simulink model "rfdc"  (R2019a)
settings: Solver=VariableStepAuto  StartTime=0.0  StopTime=10.0  RelTol=1e-3
libraries: xbsIndex_r4 x6
(part 1 of 2)
settings Model: Creator=mcb  LastModifiedBy=bjacobm

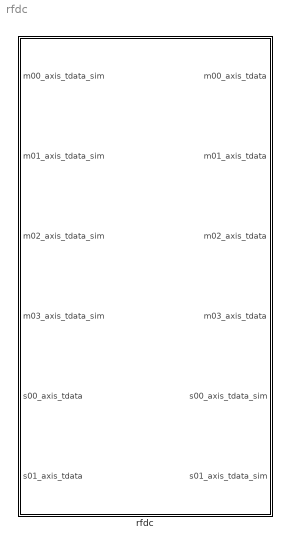
== system rfdc ==
  rfdc : Subsystem  Tag=xps:rfdc  mask(Xilinx RF Data Converter){forceredraw=0, maskopening=1, runinit=1, Tile224_enable=on, t224_enable_mts=off, t224_sample_rate=2000, t224_clk_out=125, t224_enable_pll=on, t224_ref_clk=250, t224_axi_stream_clk=[], t224_QT_adc0_enable=on, t224_QT_adc0_digital_output=I/Q, t224_QT_adc0_dec_mode=4x, t224_QT_adc0_sample_per_cycle=4, t224_QT_adc0_req_axis_clk=250, t224_QT_adc0_mixer_type=Fine, t224_QT_adc0_mixer_mode=Real -> I/Q, t224_QT_adc0_nco_freq=0, t224_QT_adc0_nco_phase=0, t224_QT_adc0_coarse_freq=0, t224_QT_adc0_nyquist_zone=Zone 1, t224_QT_adc0_cal_mode=Mode 2, t224_QT_adc1_enable=on, t224_QT_adc1_digital_output=I/Q, t224_QT_adc1_dec_mode=4x, t224_QT_adc1_sample_per_cycle=4, t224_QT_adc1_req_axis_clk=250, t224_QT_adc1_mixer_type=Fine, t224_QT_adc1_mixer_mode=Real -> I/Q, t224_QT_adc1_nco_freq=0, t224_QT_adc1_nco_phase=0, t224_QT_adc1_coarse_freq=0, t224_QT_adc1_nyquist_zone=Zone 1, t224_QT_adc1_cal_mode=Mode 2, t224_QT_adc2_enable=on, t224_QT_adc2_digital_output=I/Q, t224_QT_adc2_dec_mode=4x, t224_QT_adc2_sample_per_cycle=4, t224_QT_adc2_req_axis_clk=250, t224_QT_adc2_mixer_type=Fine, t224_QT_adc2_mixer_mode=Real -> I/Q, t224_QT_adc2_nco_freq=0, t224_QT_adc2_nco_phase=0, t224_QT_adc2_coarse_freq=0, t224_QT_adc2_nyquist_zone=Zone 1, t224_QT_adc2_cal_mode=Mode 2, t224_QT_adc3_enable=on, t224_QT_adc3_digital_output=I/Q, t224_QT_adc3_dec_mode=4x, t224_QT_adc3_sample_per_cycle=4, t224_QT_adc3_req_axis_clk=250, t224_QT_adc3_mixer_type=Fine, t224_QT_adc3_mixer_mode=Real -> I/Q, t224_QT_adc3_nco_freq=0, t224_QT_adc3_nco_phase=0, t224_QT_adc3_coarse_freq=0, t224_QT_adc3_nyquist_zone=Zone 1, t224_QT_adc3_cal_mode=Mode 2, t224_DT_adc0_enable=on, t224_DT_adc0_digital_output=Real, t224_DT_adc0_dec_mode=2x, t224_DT_adc0_sample_per_cycle=8, t224_DT_adc0_req_axis_clk=125, t224_DT_adc0_mixer_type=Bypassed, t224_DT_adc0_mixer_mode=Real -> Real, t224_DT_adc0_nco_freq=0, t224_DT_adc0_nco_phase=0, t224_DT_adc0_coarse_freq=0, t224_DT_adc0_nyquist_zone=Zone 1, t224_DT_adc0_cal_mode=Mode 2, t224_DT_adc1_enable=on, t224_DT_adc1_digital_output=Real, t224_DT_adc1_dec_mode=2x, t224_DT_adc1_sample_per_cycle=8, t224_DT_adc1_req_axis_clk=125, t224_DT_adc1_mixer_type=Bypassed, t224_DT_adc1_mixer_mode=Real -> Real, t224_DT_adc1_nco_freq=0, t224_DT_adc1_nco_phase=0, t224_DT_adc1_coarse_freq=0, t224_DT_adc1_nyquist_zone=Zone 1, t224_DT_adc1_cal_mode=Mode 2, Tile225_enable=off, t225_enable_mts=off, t225_sample_rate=2000, t225_clk_out=125, t225_enable_pll=on, t225_ref_clk=250, t225_axi_stream_clk=[], t225_QT_adc0_enable=on, t225_QT_adc0_digital_output=Real, t225_QT_adc0_dec_mode=4x, t225_QT_adc0_sample_per_cycle=2, t225_QT_adc0_req_axis_clk=250, t225_QT_adc0_mixer_type=Bypassed, t225_QT_adc0_mixer_mode=Real -> Real, t225_QT_adc0_nco_freq=0, t225_QT_adc0_nco_phase=0, t225_QT_adc0_coarse_freq=0, t225_QT_adc0_nyquist_zone=Zone 1, t225_QT_adc0_cal_mode=Mode 2, t225_QT_adc1_enable=off, t225_QT_adc1_digital_output=Real, t225_QT_adc1_dec_mode=4x, t225_QT_adc1_sample_per_cycle=2, t225_QT_adc1_req_axis_clk=250, t225_QT_adc1_mixer_type=Bypassed, t225_QT_adc1_mixer_mode=Real -> Real, t225_QT_adc1_nco_freq=0, t225_QT_adc1_nco_phase=0, t225_QT_adc1_coarse_freq=0, t225_QT_adc1_nyquist_zone=Zone 1, t225_QT_adc1_cal_mode=Mode 2, t225_QT_adc2_enable=off, t225_QT_adc2_digital_output=Real, t225_QT_adc2_dec_mode=4x, t225_QT_adc2_sample_per_cycle=2, t225_QT_adc2_req_axis_clk=250, t225_QT_adc2_mixer_type=Bypassed, t225_QT_adc2_mixer_mode=Real -> Real, t225_QT_adc2_nco_freq=0, t225_QT_adc2_nco_phase=0, t225_QT_adc2_coarse_freq=0, t225_QT_adc2_nyquist_zone=Zone 1, t225_QT_adc2_cal_mode=Mode 2, t225_QT_adc3_enable=off, t225_QT_adc3_digital_output=Real, t225_QT_adc3_dec_mode=4x, t225_QT_adc3_sample_per_cycle=2, t225_QT_adc3_req_axis_clk=250, t225_QT_adc3_mixer_type=Bypassed, t225_QT_adc3_mixer_mode=Real -> Real, t225_QT_adc3_nco_freq=0, t225_QT_adc3_nco_phase=0, t225_QT_adc3_coarse_freq=0, t225_QT_adc3_nyquist_zone=Zone 1, t225_QT_adc3_cal_mode=Mode 2, t225_DT_adc0_enable=on, t225_DT_adc0_digital_output=Real, t225_DT_adc0_dec_mode=2x, t225_DT_adc0_sample_per_cycle=8, t225_DT_adc0_req_axis_clk=125, t225_DT_adc0_mixer_type=Bypassed, t225_DT_adc0_mixer_mode=Real -> Real, t225_DT_adc0_nco_freq=0, t225_DT_adc0_nco_phase=0, t225_DT_adc0_coarse_freq=0, t225_DT_adc0_nyquist_zone=Zone 1, t225_DT_adc0_cal_mode=Mode 2, t225_DT_adc1_enable=on, t225_DT_adc1_digital_output=Real, t225_DT_adc1_dec_mode=2x, t225_DT_adc1_sample_per_cycle=8, t225_DT_adc1_req_axis_clk=125, t225_DT_adc1_mixer_type=Bypassed, t225_DT_adc1_mixer_mode=Real -> Real, t225_DT_adc1_nco_freq=0, t225_DT_adc1_nco_phase=0, t225_DT_adc1_coarse_freq=0, t225_DT_adc1_nyquist_zone=Zone 1, t225_DT_adc1_cal_mode=Mode 2, Tile226_enable=off, t226_enable_mts=off, t226_sample_rate=2000, t226_clk_out=125, t226_enable_pll=on, t226_ref_clk=250, t226_axi_stream_clk=[], t226_QT_adc0_enable=on, t226_QT_adc0_digital_output=Real, t226_QT_adc0_dec_mode=4x, t226_QT_adc0_sample_per_cycle=2, t226_QT_adc0_req_axis_clk=250, t226_QT_adc0_mixer_type=Bypassed, t226_QT_adc0_mixer_mode=Real -> Real, t226_QT_adc0_nco_freq=0, t226_QT_adc0_nco_phase=0, t226_QT_adc0_coarse_freq=0, t226_QT_adc0_nyquist_zone=Zone 1, t226_QT_adc0_cal_mode=Mode 2, t226_QT_adc1_enable=off, t226_QT_adc1_digital_output=Real, t226_QT_adc1_dec_mode=4x, t226_QT_adc1_sample_per_cycle=2, t226_QT_adc1_req_axis_clk=250, t226_QT_adc1_mixer_type=Bypassed, t226_QT_adc1_mixer_mode=Real -> Real, t226_QT_adc1_nco_freq=0, t226_QT_adc1_nco_phase=0, t226_QT_adc1_coarse_freq=0, t226_QT_adc1_nyquist_zone=Zone 1, t226_QT_adc1_cal_mode=Mode 2, t226_QT_adc2_enable=off, t226_QT_adc2_digital_output=Real, t226_QT_adc2_dec_mode=4x, t226_QT_adc2_sample_per_cycle=2, t226_QT_adc2_req_axis_clk=250, t226_QT_adc2_mixer_type=Bypassed, t226_QT_adc2_mixer_mode=Real -> Real, t226_QT_adc2_nco_freq=0, t226_QT_adc2_nco_phase=0, t226_QT_adc2_coarse_freq=0, t226_QT_adc2_nyquist_zone=Zone 1, t226_QT_adc2_cal_mode=Mode 2, t226_QT_adc3_enable=off, t226_QT_adc3_digital_output=Real, t226_QT_adc3_dec_mode=4x, t226_QT_adc3_sample_per_cycle=2, t226_QT_adc3_req_axis_clk=250, t226_QT_adc3_mixer_type=Bypassed, t226_QT_adc3_mixer_mode=Real -> Real, t226_QT_adc3_nco_freq=0, t226_QT_adc3_nco_phase=0, t226_QT_adc3_coarse_freq=0, t226_QT_adc3_nyquist_zone=Zone 1, t226_QT_adc3_cal_mode=Mode 2, t226_DT_adc0_enable=on, t226_DT_adc0_digital_output=Real, t226_DT_adc0_dec_mode=2x, t226_DT_adc0_sample_per_cycle=8, t226_DT_adc0_req_axis_clk=125, t226_DT_adc0_mixer_type=Bypassed, t226_DT_adc0_mixer_mode=Real -> Real, t226_DT_adc0_nco_freq=0, t226_DT_adc0_nco_phase=0, t226_DT_adc0_coarse_freq=0, t226_DT_adc0_nyquist_zone=Zone 1, t226_DT_adc0_cal_mode=Mode 2, t226_DT_adc1_enable=on, t226_DT_adc1_digital_output=Real, t226_DT_adc1_dec_mode=2x, t226_DT_adc1_sample_per_cycle=8, t226_DT_adc1_req_axis_clk=125, t226_DT_adc1_mixer_type=Bypassed, t226_DT_adc1_mixer_mode=Real -> Real, t226_DT_adc1_nco_freq=0, t226_DT_adc1_nco_phase=0, t226_DT_adc1_coarse_freq=0, t226_DT_adc1_nyquist_zone=Zone 1, t226_DT_adc1_cal_mode=Mode 2, Tile227_enable=off, t227_enable_mts=off, t227_sample_rate=2000, t227_clk_out=125, t227_enable_pll=on, t227_ref_clk=250, t227_axi_stream_clk=[], t227_QT_adc0_enable=on, t227_QT_adc0_digital_output=Real, t227_QT_adc0_dec_mode=4x, t227_QT_adc0_sample_per_cycle=2, t227_QT_adc0_req_axis_clk=250, t227_QT_adc0_mixer_type=Bypassed, t227_QT_adc0_mixer_mode=Real -> Real, t227_QT_adc0_nco_freq=0, t227_QT_adc0_nco_phase=0, t227_QT_adc0_coarse_freq=0, t227_QT_adc0_nyquist_zone=Zone 1, t227_QT_adc0_cal_mode=Mode 2, t227_QT_adc1_enable=off, t227_QT_adc1_digital_output=Real, t227_QT_adc1_dec_mode=4x, t227_QT_adc1_sample_per_cycle=2, t227_QT_adc1_req_axis_clk=250, t227_QT_adc1_mixer_type=Bypassed, t227_QT_adc1_mixer_mode=Real -> Real, t227_QT_adc1_nco_freq=0, t227_QT_adc1_nco_phase=0, t227_QT_adc1_coarse_freq=0, t227_QT_adc1_nyquist_zone=Zone 1, t227_QT_adc1_cal_mode=Mode 2, t227_QT_adc2_enable=off, t227_QT_adc2_digital_output=Real, t227_QT_adc2_dec_mode=4x, t227_QT_adc2_sample_per_cycle=2, t227_QT_adc2_req_axis_clk=250, t227_QT_adc2_mixer_type=Bypassed, t227_QT_adc2_mixer_mode=Real -> Real, t227_QT_adc2_nco_freq=0, t227_QT_adc2_nco_phase=0, t227_QT_adc2_coarse_freq=0, t227_QT_adc2_nyquist_zone=Zone 1, t227_QT_adc2_cal_mode=Mode 2, t227_QT_adc3_enable=off, t227_QT_adc3_digital_output=Real, t227_QT_adc3_dec_mode=4x, t227_QT_adc3_sample_per_cycle=2, t227_QT_adc3_req_axis_clk=250, t227_QT_adc3_mixer_type=Bypassed, t227_QT_adc3_mixer_mode=Real -> Real, t227_QT_adc3_nco_freq=0, t227_QT_adc3_nco_phase=0, t227_QT_adc3_coarse_freq=0, t227_QT_adc3_nyquist_zone=Zone 1, t227_QT_adc3_cal_mode=Mode 2, t227_DT_adc0_enable=on, t227_DT_adc0_digital_output=Real, t227_DT_adc0_dec_mode=2x, t227_DT_adc0_sample_per_cycle=8, t227_DT_adc0_req_axis_clk=125, t227_DT_adc0_mixer_type=Bypassed, t227_DT_adc0_mixer_mode=Real -> Real, t227_DT_adc0_nco_freq=0, t227_DT_adc0_nco_phase=0, t227_DT_adc0_coarse_freq=0, t227_DT_adc0_nyquist_zone=Zone 1, t227_DT_adc0_cal_mode=Mode 2, t227_DT_adc1_enable=on, t227_DT_adc1_digital_output=Real, t227_DT_adc1_dec_mode=2x, t227_DT_adc1_sample_per_cycle=8, t227_DT_adc1_req_axis_clk=125, t227_DT_adc1_mixer_type=Bypassed, t227_DT_adc1_mixer_mode=Real -> Real, t227_DT_adc1_nco_freq=0, t227_DT_adc1_nco_phase=0, t227_DT_adc1_coarse_freq=0, t227_DT_adc1_nyquist_zone=Zone 1, t227_DT_adc1_cal_mode=Mode 2, Tile228_enable=on, t228_enable_mts=off, t228_sample_rate=2000, t228_clk_out=125, t228_enable_pll=on, t228_ref_clk=250, t228_axi_stream_clk=[], t228_output_power=20, t228_QT_dac0_enable=on, t228_QT_dac0_analog_output=Real, t228_QT_dac0_inter_mode=4x, t228_QT_dac0_sample_per_cycle=2, t228_QT_dac0_req_axis_clk=250, t228_QT_dac0_datapath_mode=DUC 0 to Fs/2, t228_QT_dac0_mixer_type=Bypassed, t228_QT_dac0_mixer_mode=Real -> Real, t228_QT_dac0_nco_freq=0, t228_QT_dac0_nco_phase=0, t228_QT_dac0_coarse_freq=0, t228_QT_dac0_nyquist_zone=Zone 1, t228_QT_dac0_decode_mode=SNR Optimized, t228_QT_dac1_enable=on, t228_QT_dac1_analog_output=Real, t228_QT_dac1_inter_mode=4x, t228_QT_dac1_sample_per_cycle=2, t228_QT_dac1_req_axis_clk=250, t228_QT_dac1_datapath_mode=DUC 0 to Fs/2, t228_QT_dac1_mixer_type=Bypassed, t228_QT_dac1_mixer_mode=Real -> Real, t228_QT_dac1_nco_freq=0, t228_QT_dac1_nco_phase=0, t228_QT_dac1_coarse_freq=0, t228_QT_dac1_nyquist_zone=Zone 1, t228_QT_dac1_decode_mode=SNR Optimized, t228_QT_dac2_enable=off, t228_QT_dac2_analog_output=Real, t228_QT_dac2_inter_mode=4x, t228_QT_dac2_sample_per_cycle=2, t228_QT_dac2_req_axis_clk=250, t228_QT_dac2_datapath_mode=DUC 0 to Fs/2, t228_QT_dac2_mixer_type=Bypassed, t228_QT_dac2_mixer_mode=Real -> Real, t228_QT_dac2_nco_freq=0, t228_QT_dac2_nco_phase=0, t228_QT_dac2_coarse_freq=0, t228_QT_dac2_nyquist_zone=Zone 1, t228_QT_dac2_decode_mode=SNR Optimized, t228_QT_dac3_enable=off, t228_QT_dac3_analog_output=Real, t228_QT_dac3_inter_mode=4x, t228_QT_dac3_sample_per_cycle=2, t228_QT_dac3_req_axis_clk=250, t228_QT_dac3_datapath_mode=DUC 0 to Fs/2, t228_QT_dac3_mixer_type=Bypassed, t228_QT_dac3_mixer_mode=Real -> Real, t228_QT_dac3_nco_freq=0, t228_QT_dac3_nco_phase=0, t228_QT_dac3_coarse_freq=0, t228_QT_dac3_nyquist_zone=Zone 1, t228_QT_dac3_decode_mode=SNR Optimized, t228_DT_dac0_enable=on, t228_DT_dac0_analog_output=I/Q, t228_DT_dac0_inter_mode=2x, t228_DT_dac0_sample_per_cycle=8, t228_DT_dac0_req_axis_clk=125, t228_DT_dac0_mixer_type=Fine, t228_DT_dac0_mixer_mode=I/Q -> I/Q, t228_DT_dac0_nco_freq=0, t228_DT_dac0_nco_phase=0, t228_DT_dac0_coarse_freq=0, t228_DT_dac0_nyquist_zone=Zone 1, t228_DT_dac0_decode_mode=SNR Optimized, t228_DT_dac1_enable=on, t228_DT_dac1_analog_output=I/Q, t228_DT_dac1_inter_mode=2x, t228_DT_dac1_sample_per_cycle=8, t228_DT_dac1_req_axis_clk=125, t228_DT_dac1_mixer_type=Off, t228_DT_dac1_mixer_mode=Off, t228_DT_dac1_nco_freq=0, t228_DT_dac1_nco_phase=0, t228_DT_dac1_coarse_freq=0, t228_DT_dac1_nyquist_zone=Zone 1, t228_DT_dac1_decode_mode=SNR Optimized, t228_DT_dac2_enable=on, t228_DT_dac2_analog_output=Real, t228_DT_dac2_inter_mode=2x, t228_DT_dac2_sample_per_cycle=8, t228_DT_dac2_req_axis_clk=125, t228_DT_dac2_mixer_type=Bypassed, t228_DT_dac2_mixer_mode=Real -> Real, t228_DT_dac2_nco_freq=0, t228_DT_dac2_nco_phase=0, t228_DT_dac2_coarse_freq=0, t228_DT_dac2_nyquist_zone=Zone 1, t228_DT_dac2_decode_mode=SNR Optimized, t228_DT_dac3_enable=off, t228_DT_dac3_analog_output=Real, t228_DT_dac3_inter_mode=2x, t228_DT_dac3_sample_per_cycle=8, t228_DT_dac3_req_axis_clk=125, t228_DT_dac3_mixer_type=Bypassed, t228_DT_dac3_mixer_mode=Real -> Real, t228_DT_dac3_nco_freq=0, t228_DT_dac3_nco_phase=0, t228_DT_dac3_coarse_freq=0, t228_DT_dac3_nyquist_zone=Zone 1, t228_DT_dac3_decode_mode=SNR Optimized, Tile229_enable=off, t229_enable_mts=off, t229_sample_rate=2000, t229_clk_out=125, t229_enable_pll=on, t229_ref_clk=250, t229_axi_stream_clk=[], t229_output_power=20, t229_QT_dac0_enable=on, t229_QT_dac0_analog_output=Real, t229_QT_dac0_inter_mode=4x, t229_QT_dac0_sample_per_cycle=2, t229_QT_dac0_req_axis_clk=250, t229_QT_dac0_datapath_mode=DUC 0 to Fs/2, t229_QT_dac0_mixer_type=Bypassed, t229_QT_dac0_mixer_mode=Real -> Real, t229_QT_dac0_nco_freq=0, t229_QT_dac0_nco_phase=0, t229_QT_dac0_coarse_freq=0, t229_QT_dac0_nyquist_zone=Zone 1, t229_QT_dac0_decode_mode=SNR Optimized, t229_QT_dac1_enable=off, t229_QT_dac1_analog_output=Real, t229_QT_dac1_inter_mode=4x, t229_QT_dac1_sample_per_cycle=2, t229_QT_dac1_req_axis_clk=250, t229_QT_dac1_datapath_mode=DUC 0 to Fs/2, t229_QT_dac1_mixer_type=Bypassed, t229_QT_dac1_mixer_mode=Real -> Real, t229_QT_dac1_nco_freq=0, t229_QT_dac1_nco_phase=0, t229_QT_dac1_coarse_freq=0, t229_QT_dac1_nyquist_zone=Zone 1, t229_QT_dac1_decode_mode=SNR Optimized, t229_QT_dac2_enable=off, t229_QT_dac2_analog_output=Real, t229_QT_dac2_inter_mode=4x, t229_QT_dac2_sample_per_cycle=2, t229_QT_dac2_req_axis_clk=250, t229_QT_dac2_datapath_mode=DUC 0 to Fs/2, t229_QT_dac2_mixer_type=Bypassed, t229_QT_dac2_mixer_mode=Real -> Real, t229_QT_dac2_nco_freq=0, t229_QT_dac2_nco_phase=0, t229_QT_dac2_coarse_freq=0, t229_QT_dac2_nyquist_zone=Zone 1, t229_QT_dac2_decode_mode=SNR Optimized, t229_QT_dac3_enable=off, t229_QT_dac3_analog_output=Real, t229_QT_dac3_inter_mode=4x, t229_QT_dac3_sample_per_cycle=2, t229_QT_dac3_req_axis_clk=250, t229_QT_dac3_datapath_mode=DUC 0 to Fs/2, t229_QT_dac3_mixer_type=Bypassed, t229_QT_dac3_mixer_mode=Real -> Real, t229_QT_dac3_nco_freq=0, t229_QT_dac3_nco_phase=0, t229_QT_dac3_coarse_freq=0, t229_QT_dac3_nyquist_zone=Zone 1, t229_QT_dac3_decode_mode=SNR Optimized, t229_DT_dac0_enable=off, t229_DT_dac0_analog_output=Real, t229_DT_dac0_inter_mode=2x, t229_DT_dac0_sample_per_cycle=8, t229_DT_dac0_req_axis_clk=125, t229_DT_dac0_mixer_type=Bypassed, t229_DT_dac0_mixer_mode=Real -> Real, t229_DT_dac0_nco_freq=0, t229_DT_dac0_nco_phase=0, t229_DT_dac0_coarse_freq=0, t229_DT_dac0_nyquist_zone=Zone 1, t229_DT_dac0_decode_mode=SNR Optimized, t229_DT_dac1_enable=off, t229_DT_dac1_analog_output=Real, t229_DT_dac1_inter_mode=2x, t229_DT_dac1_sample_per_cycle=8, t229_DT_dac1_req_axis_clk=125, t229_DT_dac1_mixer_type=Bypassed, t229_DT_dac1_mixer_mode=Real -> Real, t229_DT_dac1_nco_freq=0, t229_DT_dac1_nco_phase=0, t229_DT_dac1_coarse_freq=0, t229_DT_dac1_nyquist_zone=Zone 1, t229_DT_dac1_decode_mode=SNR Optimized, t229_DT_dac2_enable=off, t229_DT_dac2_analog_output=Real, t229_DT_dac2_inter_mode=2x, t229_DT_dac2_sample_per_cycle=8, t229_DT_dac2_req_axis_clk=125, t229_DT_dac2_mixer_type=Bypassed, t229_DT_dac2_mixer_mode=Real -> Real, t229_DT_dac2_nco_freq=0, t229_DT_dac2_nco_phase=0, t229_DT_dac2_coarse_freq=0, t229_DT_dac2_nyquist_zone=Zone 1, t229_DT_dac2_decode_mode=SNR Optimized, t229_DT_dac3_enable=off, t229_DT_dac3_analog_output=Real, t229_DT_dac3_inter_mode=2x, t229_DT_dac3_sample_per_cycle=8, t229_DT_dac3_req_axis_clk=125, t229_DT_dac3_mixer_type=Bypassed, t229_DT_dac3_mixer_mode=Real -> Real, t229_DT_dac3_nco_freq=0, t229_DT_dac3_nco_phase=0, t229_DT_dac3_coarse_freq=0, t229_DT_dac3_nyquist_zone=Zone 1, t229_DT_dac3_decode_mode=SNR Optimized, Tile230_enable=off, t230_enable_mts=off, t230_sample_rate=2000, t230_clk_out=125, t230_enable_pll=on, t230_ref_clk=250, t230_axi_stream_clk=[], t230_output_power=20, t230_QT_dac0_enable=on, t230_QT_dac0_analog_output=Real, t230_QT_dac0_inter_mode=4x, t230_QT_dac0_sample_per_cycle=2, t230_QT_dac0_req_axis_clk=250, t230_QT_dac0_datapath_mode=DUC 0 to Fs/2, t230_QT_dac0_mixer_type=Bypassed, t230_QT_dac0_mixer_mode=Real -> Real, t230_QT_dac0_nco_freq=0, t230_QT_dac0_nco_phase=0, t230_QT_dac0_coarse_freq=0, t230_QT_dac0_nyquist_zone=Zone 1, t230_QT_dac0_decode_mode=SNR Optimized, t230_QT_dac1_enable=off, t230_QT_dac1_analog_output=Real, t230_QT_dac1_inter_mode=4x, t230_QT_dac1_sample_per_cycle=2, t230_QT_dac1_req_axis_clk=250, t230_QT_dac1_datapath_mode=DUC 0 to Fs/2, t230_QT_dac1_mixer_type=Bypassed, t230_QT_dac1_mixer_mode=Real -> Real, t230_QT_dac1_nco_freq=0, t230_QT_dac1_nco_phase=0, t230_QT_dac1_coarse_freq=0, t230_QT_dac1_nyquist_zone=Zone 1, t230_QT_dac1_decode_mode=SNR Optimized, t230_QT_dac2_enable=off, t230_QT_dac2_analog_output=Real, t230_QT_dac2_inter_mode=4x, t230_QT_dac2_sample_per_cycle=2, t230_QT_dac2_req_axis_clk=250, t230_QT_dac2_datapath_mode=DUC 0 to Fs/2, t230_QT_dac2_mixer_type=Bypassed, t230_QT_dac2_mixer_mode=Real -> Real, t230_QT_dac2_nco_freq=0, t230_QT_dac2_nco_phase=0, t230_QT_dac2_coarse_freq=0, t230_QT_dac2_nyquist_zone=Zone 1, t230_QT_dac2_decode_mode=SNR Optimized, t230_QT_dac3_enable=off, t230_QT_dac3_analog_output=Real, t230_QT_dac3_inter_mode=4x, t230_QT_dac3_sample_per_cycle=2, t230_QT_dac3_req_axis_clk=250, t230_QT_dac3_datapath_mode=DUC 0 to Fs/2, t230_QT_dac3_mixer_type=Bypassed, t230_QT_dac3_mixer_mode=Real -> Real, t230_QT_dac3_nco_freq=0, t230_QT_dac3_nco_phase=0, t230_QT_dac3_coarse_freq=0, t230_QT_dac3_nyquist_zone=Zone 1, t230_QT_dac3_decode_mode=SNR Optimized, Tile231_enable=off, t231_enable_mts=off, t231_sample_rate=2000, t231_clk_out=125, t231_enable_pll=on, t231_ref_clk=250, t231_axi_stream_clk=[], t231_output_power=20, t231_QT_dac0_enable=on, t231_QT_dac0_analog_output=Real, t231_QT_dac0_inter_mode=4x, t231_QT_dac0_sample_per_cycle=2, t231_QT_dac0_req_axis_clk=250, t231_QT_dac0_datapath_mode=DUC 0 to Fs/2, t231_QT_dac0_mixer_type=Bypassed, t231_QT_dac0_mixer_mode=Real -> Real, t231_QT_dac0_nco_freq=0, t231_QT_dac0_nco_phase=0, t231_QT_dac0_coarse_freq=0, t231_QT_dac0_nyquist_zone=Zone 1, t231_QT_dac0_decode_mode=SNR Optimized, t231_QT_dac1_enable=off, t231_QT_dac1_analog_output=Real, t231_QT_dac1_inter_mode=4x, t231_QT_dac1_sample_per_cycle=2, t231_QT_dac1_req_axis_clk=250, t231_QT_dac1_datapath_mode=DUC 0 to Fs/2, t231_QT_dac1_mixer_type=Bypassed, t231_QT_dac1_mixer_mode=Real -> Real, t231_QT_dac1_nco_freq=0, t231_QT_dac1_nco_phase=0, t231_QT_dac1_coarse_freq=0, t231_QT_dac1_nyquist_zone=Zone 1, t231_QT_dac1_decode_mode=SNR Optimized, t231_QT_dac2_enable=off, t231_QT_dac2_analog_output=Real, t231_QT_dac2_inter_mode=4x, t231_QT_dac2_sample_per_cycle=2, t231_QT_dac2_req_axis_clk=250, t231_QT_dac2_datapath_mode=DUC 0 to Fs/2, t231_QT_dac2_mixer_type=Bypassed, t231_QT_dac2_mixer_mode=Real -> Real, t231_QT_dac2_nco_freq=0, t231_QT_dac2_nco_phase=0, t231_QT_dac2_coarse_freq=0, t231_QT_dac2_nyquist_zone=Zone 1, t231_QT_dac2_decode_mode=SNR Optimized, t231_QT_dac3_enable=off, t231_QT_dac3_analog_output=Real, t231_QT_dac3_inter_mode=4x, t231_QT_dac3_sample_per_cycle=2, t231_QT_dac3_req_axis_clk=250, t231_QT_dac3_datapath_mode=DUC 0 to Fs/2, t231_QT_dac3_mixer_type=Bypassed, t231_QT_dac3_mixer_mode=Real -> Real, t231_QT_dac3_nco_freq=0, t231_QT_dac3_nco_phase=0, t231_QT_dac3_coarse_freq=0, t231_QT_dac3_nyquist_zone=Zone 1, t231_QT_dac3_decode_mode=SNR Optimized, t224_has_adc_clk=off, t224_adc_clk_src=226, t224_clk_dist=None, t225_has_adc_clk=on, t225_adc_clk_src=226, t225_clk_dist=None, t226_has_adc_clk=on, t226_adc_clk_src=226, t226_clk_dist=Input Refclk, t227_has_adc_clk=off, t227_adc_clk_src=226, t227_clk_dist=None, t228_has_dac_clk=off, t228_dac_clk_src=230, t228_clk_dist=None, t229_has_dac_clk=on, t229_dac_clk_src=230, t229_clk_dist=None, t230_has_dac_clk=on, t230_dac_clk_src=230, t230_clk_dist=Input Refclk, t231_has_dac_clk=off, t231_dac_clk_src=230, t231_clk_dist=None, maskdoneopening=0}
      mask prompts: Tile224_enable "Enable Tile"; t224_enable_mts "Enable Multi-Tile Sync"; t224_sample_rate "Sampling Rate (Msps)"; t224_clk_out "Clock Out (MHz)"; t224_enable_pll "Enable Tile PLLs"; t224_ref_clk "Reference Clock (MHz)"; t224_axi_stream_clk "Required AXI4-Stream Clock (MHz)"; t224_QT_adc0_enable "Enable ADC"; t224_QT_adc0_digital_output "Digital Output Data"; t224_QT_adc0_dec_mode "Decimation Mode"; t224_QT_adc0_sample_per_cycle "Samples per AXI4-Stream Cycle"; t224_QT_adc0_mixer_type "Mixer Type"; t224_QT_adc0_mixer_mode "Mixer Mode"; t224_QT_adc0_nco_freq "NCO Frequency (GHz)"; t224_QT_adc0_nco_phase "NCO Phase"; t224_QT_adc0_coarse_freq "Frequency"; t224_QT_adc0_nyquist_zone "Nyquist Zone"; t224_QT_adc0_cal_mode "Calibration Mode"; t224_QT_adc1_enable "Enable ADC"; t224_QT_adc1_digital_output "Digital Output Data"; t224_QT_adc1_dec_mode "Decimation Mode"; t224_QT_adc1_sample_per_cycle "Samples per AXI4-Stream Cycle"; t224_QT_adc1_mixer_type "Mixer Type"; t224_QT_adc1_mixer_mode "Mixer Mode"; t224_QT_adc1_nco_freq "NCO Frequency (GHz)"; t224_QT_adc1_nco_phase "NCO Phase"; t224_QT_adc1_coarse_freq "Frequency"; t224_QT_adc1_nyquist_zone "Nyquist Zone"; t224_QT_adc1_cal_mode "Calibration Mode"; t224_QT_adc2_enable "Enable ADC"; t224_QT_adc2_digital_output "Digital Output Data"; t224_QT_adc2_dec_mode "Decimation Mode"; t224_QT_adc2_sample_per_cycle "Samples per AXI4-Stream Cycle"; t224_QT_adc2_mixer_type "Mixer Type"; t224_QT_adc2_mixer_mode "Mixer Mode"; t224_QT_adc2_nco_freq "NCO Frequency (GHz)"; t224_QT_adc2_nco_phase "NCO Phase"; t224_QT_adc2_coarse_freq "Frequency"; t224_QT_adc2_nyquist_zone "Nyquist Zone"; t224_QT_adc2_cal_mode "Calibration Mode"; t224_QT_adc3_enable "Enable ADC"; t224_QT_adc3_digital_output "Digital Output Data"; t224_QT_adc3_dec_mode "Decimation Mode"; t224_QT_adc3_sample_per_cycle "Samples per AXI4-Stream Cycle"; t224_QT_adc3_mixer_type "Mixer Type"; t224_QT_adc3_mixer_mode "Mixer Mode"; t224_QT_adc3_nco_freq "NCO Frequency (GHz)"; t224_QT_adc3_nco_phase "NCO Phase"; t224_QT_adc3_coarse_freq "Frequency"; t224_QT_adc3_nyquist_zone "Nyquist Zone"; t224_QT_adc3_cal_mode "Calibration Mode"; t224_DT_adc0_enable "Enable ADC"; t224_DT_adc0_digital_output "Digital Output Data"; t224_DT_adc0_dec_mode "Decimation Mode"; t224_DT_adc0_sample_per_cycle "Samples per AXI4-Stream Cycle"; t224_DT_adc0_mixer_type "Mixer Type"; t224_DT_adc0_mixer_mode "Mixer Mode"; t224_DT_adc0_nco_freq "NCO Frequency (GHz)"; t224_DT_adc0_nco_phase "NCO Phase"; t224_DT_adc0_coarse_freq "Frequency"; t224_DT_adc0_nyquist_zone "Nyquist Zone"; t224_DT_adc0_cal_mode "Calibration Mode"; t224_DT_adc1_enable "Enable ADC"; t224_DT_adc1_digital_output "Digital Output Data"; t224_DT_adc1_dec_mode "Decimation Mode"; t224_DT_adc1_sample_per_cycle "Samples per AXI4-Stream Cycle"; t224_DT_adc1_mixer_type "Mixer Type"; t224_DT_adc1_mixer_mode "Mixer Mode"; t224_DT_adc1_nco_freq "NCO Frequency (GHz)"; t224_DT_adc1_nco_phase "NCO Phase"; t224_DT_adc1_coarse_freq "Frequency"; t224_DT_adc1_nyquist_zone "Nyquist Zone"; t224_DT_adc1_cal_mode "Calibration Mode"; Tile225_enable "Enable Tile"; t225_enable_mts "Enable Multi-Tile Sync"; t225_sample_rate "Sampling Rate (Msps)"; t225_clk_out "Clock Out (MHz)"; t225_enable_pll "Enable Tile PLLs"; t225_ref_clk "Reference Clock (MHz)"; t225_axi_stream_clk "Required AXI4-Stream Clock (MHz)"; t225_QT_adc0_enable "Enable ADC"; t225_QT_adc0_digital_output "Digital Output Data"; t225_QT_adc0_dec_mode "Decimation Mode"; t225_QT_adc0_sample_per_cycle "Samples per AXI4-Stream Cycle"; t225_QT_adc0_mixer_type "Mixer Type"; t225_QT_adc0_mixer_mode "Mixer Mode"; t225_QT_adc0_nco_freq "NCO Frequency (GHz)"; t225_QT_adc0_nco_phase "NCO Phase"; t225_QT_adc0_coarse_freq "Frequency"; t225_QT_adc0_nyquist_zone "Nyquist Zone"; t225_QT_adc0_cal_mode "Calibration Mode"; t225_QT_adc1_enable "Enable ADC"; t225_QT_adc1_digital_output "Digital Output Data"; t225_QT_adc1_dec_mode "Decimation Mode"; t225_QT_adc1_sample_per_cycle "Samples per AXI4-Stream Cycle"; t225_QT_adc1_mixer_type "Mixer Type"; t225_QT_adc1_mixer_mode "Mixer Mode"; t225_QT_adc1_nco_freq "NCO Frequency (GHz)"; t225_QT_adc1_nco_phase "NCO Phase"; t225_QT_adc1_coarse_freq "Frequency"; t225_QT_adc1_nyquist_zone "Nyquist Zone"; t225_QT_adc1_cal_mode "Calibration Mode"; t225_QT_adc2_enable "Enable ADC"; t225_QT_adc2_digital_output "Digital Output Data"; t225_QT_adc2_dec_mode "Decimation Mode"; t225_QT_adc2_sample_per_cycle "Samples per AXI4-Stream Cycle"; t225_QT_adc2_mixer_type "Mixer Type"; t225_QT_adc2_mixer_mode "Mixer Mode"; t225_QT_adc2_nco_freq "NCO Frequency (GHz)"; t225_QT_adc2_nco_phase "NCO Phase"; t225_QT_adc2_coarse_freq "Frequency"; t225_QT_adc2_nyquist_zone "Nyquist Zone"; t225_QT_adc2_cal_mode "Calibration Mode"; t225_QT_adc3_enable "Enable ADC"; t225_QT_adc3_digital_output "Digital Output Data"; t225_QT_adc3_dec_mode "Decimation Mode"; t225_QT_adc3_sample_per_cycle "Samples per AXI4-Stream Cycle"; t225_QT_adc3_mixer_type "Mixer Type"; t225_QT_adc3_mixer_mode "Mixer Mode"; t225_QT_adc3_nco_freq "NCO Frequency (GHz)"; t225_QT_adc3_nco_phase "NCO Phase"; t225_QT_adc3_coarse_freq "Frequency"; t225_QT_adc3_nyquist_zone "Nyquist Zone"; t225_QT_adc3_cal_mode "Calibration Mode"; t225_DT_adc0_enable "Enable ADC"; t225_DT_adc0_digital_output "Digital Output Data"; t225_DT_adc0_dec_mode "Decimation Mode"; t225_DT_adc0_sample_per_cycle "Samples per AXI4-Stream Cycle"; t225_DT_adc0_mixer_type "Mixer Type"; t225_DT_adc0_mixer_mode "Mixer Mode"; t225_DT_adc0_nco_freq "NCO Frequency (GHz)"; t225_DT_adc0_nco_phase "NCO Phase"; t225_DT_adc0_coarse_freq "Frequency"; t225_DT_adc0_nyquist_zone "Nyquist Zone"; t225_DT_adc0_cal_mode "Calibration Mode"; t225_DT_adc1_enable "Enable ADC"; t225_DT_adc1_digital_output "Digital Output Data"; t225_DT_adc1_dec_mode "Decimation Mode"; t225_DT_adc1_sample_per_cycle "Samples per AXI4-Stream Cycle"; t225_DT_adc1_mixer_type "Mixer Type"; t225_DT_adc1_mixer_mode "Mixer Mode"; t225_DT_adc1_nco_freq "NCO Frequency (GHz)"; t225_DT_adc1_nco_phase "NCO Phase"; t225_DT_adc1_coarse_freq "Frequency"; t225_DT_adc1_nyquist_zone "Nyquist Zone"; t225_DT_adc1_cal_mode "Calibration Mode"; Tile226_enable "Enable Tile"; t226_enable_mts "Enable Multi-Tile Sync"; t226_sample_rate "Sampling Rate (Msps)"; t226_clk_out "Clock Out (MHz)"; t226_enable_pll "Enable Tile PLLs"; t226_ref_clk "Reference Clock (MHz)"; t226_axi_stream_clk "Required AXI4-Stream Clock (MHz)"; t226_QT_adc0_enable "Enable ADC"; t226_QT_adc0_digital_output "Digital Output Data"; t226_QT_adc0_dec_mode "Decimation Mode"; t226_QT_adc0_sample_per_cycle "Samples per AXI4-Stream Cycle"; t226_QT_adc0_mixer_type "Mixer Type"; t226_QT_adc0_mixer_mode "Mixer Mode"; t226_QT_adc0_nco_freq "NCO Frequency (GHz)"; t226_QT_adc0_nco_phase "NCO Phase"; t226_QT_adc0_coarse_freq "Frequency"; t226_QT_adc0_nyquist_zone "Nyquist Zone"; t226_QT_adc0_cal_mode "Calibration Mode"; t226_QT_adc1_enable "Enable ADC"; t226_QT_adc1_digital_output "Digital Output Data"; t226_QT_adc1_dec_mode "Decimation Mode"; t226_QT_adc1_sample_per_cycle "Samples per AXI4-Stream Cycle"; t226_QT_adc1_mixer_type "Mixer Type"; t226_QT_adc1_mixer_mode "Mixer Mode"; t226_QT_adc1_nco_freq "NCO Frequency (GHz)"; t226_QT_adc1_nco_phase "NCO Phase"; t226_QT_adc1_coarse_freq "Frequency"; t226_QT_adc1_nyquist_zone "Nyquist Zone"; t226_QT_adc1_cal_mode "Calibration Mode"; t226_QT_adc2_enable "Enable ADC"; t226_QT_adc2_digital_output "Digital Output Data"; t226_QT_adc2_dec_mode "Decimation Mode"; t226_QT_adc2_sample_per_cycle "Samples per AXI4-Stream Cycle"; t226_QT_adc2_mixer_type "Mixer Type"; t226_QT_adc2_mixer_mode "Mixer Mode"; t226_QT_adc2_nco_freq "NCO Frequency (GHz)"; t226_QT_adc2_nco_phase "NCO Phase"; t226_QT_adc2_coarse_freq "Frequency"; t226_QT_adc2_nyquist_zone "Nyquist Zone"; t226_QT_adc2_cal_mode "Calibration Mode"; t226_QT_adc3_enable "Enable ADC"; t226_QT_adc3_digital_output "Digital Output Data"; t226_QT_adc3_dec_mode "Decimation Mode"; t226_QT_adc3_sample_per_cycle "Samples per AXI4-Stream Cycle"; t226_QT_adc3_mixer_type "Mixer Type"; t226_QT_adc3_mixer_mode "Mixer Mode"; t226_QT_adc3_nco_freq "NCO Frequency (GHz)"; t226_QT_adc3_nco_phase "NCO Phase"; t226_QT_adc3_coarse_freq "Frequency"; t226_QT_adc3_nyquist_zone "Nyquist Zone"; t226_QT_adc3_cal_mode "Calibration Mode"; t226_DT_adc0_enable "Enable ADC"; t226_DT_adc0_digital_output "Digital Output Data"; t226_DT_adc0_dec_mode "Decimation Mode"; t226_DT_adc0_sample_per_cycle "Samples per AXI4-Stream Cycle"; t226_DT_adc0_mixer_type "Mixer Type"; t226_DT_adc0_mixer_mode "Mixer Mode"; t226_DT_adc0_nco_freq "NCO Frequency (GHz)"; t226_DT_adc0_nco_phase "NCO Phase"; t226_DT_adc0_coarse_freq "Frequency"; t226_DT_adc0_nyquist_zone "Nyquist Zone"; t226_DT_adc0_cal_mode "Calibration Mode"; t226_DT_adc1_enable "Enable ADC"; t226_DT_adc1_digital_output "Digital Output Data"; t226_DT_adc1_dec_mode "Decimation Mode"; t226_DT_adc1_sample_per_cycle "Samples per AXI4-Stream Cycle"; t226_DT_adc1_mixer_type "Mixer Type"; t226_DT_adc1_mixer_mode "Mixer Mode"; t226_DT_adc1_nco_freq "NCO Frequency (GHz)"; t226_DT_adc1_nco_phase "NCO Phase"; t226_DT_adc1_coarse_freq "Frequency"; t226_DT_adc1_nyquist_zone "Nyquist Zone"; t226_DT_adc1_cal_mode "Calibration Mode"; Tile227_enable "Enable Tile"; t227_enable_mts "Enable Multi-Tile Sync"; t227_sample_rate "Sampling Rate (Msps)"; t227_clk_out "Clock Out (MHz)"; t227_enable_pll "Enable Tile PLLs"; t227_ref_clk "Reference Clock (MHz)"; t227_axi_stream_clk "Required AXI4-Stream Clock (MHz)"; t227_QT_adc0_enable "Enable ADC"; t227_QT_adc0_digital_output "Digital Output Data"; t227_QT_adc0_dec_mode "Decimation Mode"; t227_QT_adc0_sample_per_cycle "Samples per AXI4-Stream Cycle"; t227_QT_adc0_mixer_type "Mixer Type"; t227_QT_adc0_mixer_mode "Mixer Mode"; t227_QT_adc0_nco_freq "NCO Frequency (GHz)"; t227_QT_adc0_nco_phase "NCO Phase"; t227_QT_adc0_coarse_freq "Frequency"; t227_QT_adc0_nyquist_zone "Nyquist Zone"; t227_QT_adc0_cal_mode "Calibration Mode"; t227_QT_adc1_enable "Enable ADC"; t227_QT_adc1_digital_output "Digital Output Data"; t227_QT_adc1_dec_mode "Decimation Mode"; t227_QT_adc1_sample_per_cycle "Samples per AXI4-Stream Cycle"; t227_QT_adc1_mixer_type "Mixer Type"; t227_QT_adc1_mixer_mode "Mixer Mode"; t227_QT_adc1_nco_freq "NCO Frequency (GHz)"; t227_QT_adc1_nco_phase "NCO Phase"; t227_QT_adc1_coarse_freq "Frequency"; t227_QT_adc1_nyquist_zone "Nyquist Zone"; t227_QT_adc1_cal_mode "Calibration Mode"; t227_QT_adc2_enable "Enable ADC"; t227_QT_adc2_digital_output "Digital Output Data"; t227_QT_adc2_dec_mode "Decimation Mode"; t227_QT_adc2_sample_per_cycle "Samples per AXI4-Stream Cycle"; t227_QT_adc2_mixer_type "Mixer Type"; t227_QT_adc2_mixer_mode "Mixer Mode"; t227_QT_adc2_nco_freq "NCO Frequency (GHz)"; t227_QT_adc2_nco_phase "NCO Phase"; t227_QT_adc2_coarse_freq "Frequency"; t227_QT_adc2_nyquist_zone "Nyquist Zone"; t227_QT_adc2_cal_mode "Calibration Mode"; t227_QT_adc3_enable "Enable ADC"; t227_QT_adc3_digital_output "Digital Output Data"; t227_QT_adc3_dec_mode "Decimation Mode"; t227_QT_adc3_sample_per_cycle "Samples per AXI4-Stream Cycle"; t227_QT_adc3_mixer_type "Mixer Type"; t227_QT_adc3_mixer_mode "Mixer Mode"; t227_QT_adc3_nco_freq "NCO Frequency (GHz)"; t227_QT_adc3_nco_phase "NCO Phase"; t227_QT_adc3_coarse_freq "Frequency"; t227_QT_adc3_nyquist_zone "Nyquist Zone"; t227_QT_adc3_cal_mode "Calibration Mode"; t227_DT_adc0_enable "Enable ADC"; t227_DT_adc0_digital_output "Digital Output Data"; t227_DT_adc0_dec_mode "Decimation Mode"; t227_DT_adc0_sample_per_cycle "Samples per AXI4-Stream Cycle"; t227_DT_adc0_mixer_type "Mixer Type"; t227_DT_adc0_mixer_mode "Mixer Mode"; t227_DT_adc0_nco_freq "NCO Frequency (GHz)"; t227_DT_adc0_nco_phase "NCO Phase"; t227_DT_adc0_coarse_freq "Frequency"; t227_DT_adc0_nyquist_zone "Nyquist Zone"; t227_DT_adc0_cal_mode "Calibration Mode"; t227_DT_adc1_enable "Enable ADC"; t227_DT_adc1_digital_output "Digital Output Data"; t227_DT_adc1_dec_mode "Decimation Mode"; t227_DT_adc1_sample_per_cycle "Samples per AXI4-Stream Cycle"; t227_DT_adc1_mixer_type "Mixer Type"; t227_DT_adc1_mixer_mode "Mixer Mode"; t227_DT_adc1_nco_freq "NCO Frequency (GHz)"; t227_DT_adc1_nco_phase "NCO Phase"; t227_DT_adc1_coarse_freq "Frequency"; t227_DT_adc1_nyquist_zone "Nyquist Zone"; t227_DT_adc1_cal_mode "Calibration Mode"; Tile228_enable "Enable Tile"; t228_enable_mts "Enable Multi-Tile Sync"; t228_sample_rate "Sampling Rate (Msps)"; t228_clk_out "Clock Out (MHz)"; t228_enable_pll "Enable Tile PLLs"; t228_ref_clk "Reference Clock (MHz)"; t228_axi_stream_clk "Required AXI4-Stream Clock (MHz)"; t228_output_power "Output Power"; t228_QT_dac0_enable "Enable DAC"; t228_QT_dac0_analog_output "Analog Output Data"; t228_QT_dac0_inter_mode "Interpolation Mode"; t228_QT_dac0_sample_per_cycle "Samples per AXI4-Stream Cycle"; t228_QT_dac0_datapath_mode "Datapath Mode"; t228_QT_dac0_mixer_type "Mixer Type"; t228_QT_dac0_mixer_mode "Mixer Mode"; t228_QT_dac0_nco_freq "NCO Frequency (GHz)"; t228_QT_dac0_nco_phase "NCO Phase"; t228_QT_dac0_coarse_freq "Frequency"; t228_QT_dac0_nyquist_zone "Nyquist Zone"; t228_QT_dac0_decode_mode "Decoder Mode"; t228_QT_dac1_enable "Enable DAC"; t228_QT_dac1_analog_output "Analog Output Data"; t228_QT_dac1_inter_mode "Interpolation Mode"; t228_QT_dac1_sample_per_cycle "Samples per AXI4-Stream Cycle"; t228_QT_dac1_datapath_mode "Datapath Mode"; t228_QT_dac1_mixer_type "Mixer Type"; t228_QT_dac1_mixer_mode "Mixer Mode"; t228_QT_dac1_nco_freq "NCO Frequency (GHz)"; t228_QT_dac1_nco_phase "NCO Phase"; t228_QT_dac1_coarse_freq "Frequency"; t228_QT_dac1_nyquist_zone "Nyquist Zone"; t228_QT_dac1_decode_mode "Decoder Mode"; t228_QT_dac2_enable "Enable DAC"; t228_QT_dac2_analog_output "Analog Output Data"; t228_QT_dac2_inter_mode "Interpolation Mode"; t228_QT_dac2_sample_per_cycle "Samples per AXI4-Stream Cycle"; t228_QT_dac2_datapath_mode "Datapath Mode"; t228_QT_dac2_mixer_type "Mixer Type"; t228_QT_dac2_mixer_mode "Mixer Mode"; t228_QT_dac2_nco_freq "NCO Frequency (GHz)"; t228_QT_dac2_nco_phase "NCO Phase"; t228_QT_dac2_coarse_freq "Frequency"; t228_QT_dac2_nyquist_zone "Nyquist Zone"; t228_QT_dac2_decode_mode "Decoder Mode"; t228_QT_dac3_enable "Enable DAC"; t228_QT_dac3_analog_output "Analog Output Data"; t228_QT_dac3_inter_mode "Interpolation Mode"; t228_QT_dac3_sample_per_cycle "Samples per AXI4-Stream Cycle"; t228_QT_dac3_datapath_mode "Datapath Mode"; t228_QT_dac3_mixer_type "Mixer Type"; t228_QT_dac3_mixer_mode "Mixer Mode"; t228_QT_dac3_nco_freq "NCO Frequency (GHz)"; t228_QT_dac3_nco_phase "NCO Phase"; t228_QT_dac3_coarse_freq "Frequency"; t228_QT_dac3_nyquist_zone "Nyquist Zone"; t228_QT_dac3_decode_mode "Decoder Mode"; t228_DT_dac0_enable "Enable DAC"; t228_DT_dac0_analog_output "Analog Output Data"; t228_DT_dac0_inter_mode "Interpolation Mode"; t228_DT_dac0_sample_per_cycle "Samples per AXI4-Stream Cycle"; t228_DT_dac0_mixer_type "Mixer Type"; t228_DT_dac0_mixer_mode "Mixer Mode"; t228_DT_dac0_nco_freq "NCO Frequency (GHz)"; t228_DT_dac0_nco_phase "NCO Phase"; t228_DT_dac0_coarse_freq "Frequency"; t228_DT_dac0_nyquist_zone "Nyquist Zone"; t228_DT_dac0_decode_mode "Decoder Mode"; t228_DT_dac1_enable "Enable DAC"; t228_DT_dac1_analog_output "Analog Output Data"; t228_DT_dac1_inter_mode "Interpolation Mode"; t228_DT_dac1_sample_per_cycle "Samples per AXI4-Stream Cycle"; t228_DT_dac1_mixer_type "Mixer Type"; t228_DT_dac1_mixer_mode "Mixer Mode"; t228_DT_dac1_nco_freq "NCO Frequency (GHz)"; t228_DT_dac1_nco_phase "NCO Phase"; t228_DT_dac1_coarse_freq "Frequency"; t228_DT_dac1_nyquist_zone "Nyquist Zone"; t228_DT_dac1_decode_mode "Decoder Mode"; t228_DT_dac2_enable "Enable DAC"; t228_DT_dac2_analog_output "Analog Output Data"; t228_DT_dac2_inter_mode "Interpolation Mode"; t228_DT_dac2_sample_per_cycle "Samples per AXI4-Stream Cycle"; t228_DT_dac2_mixer_type "Mixer Type"; t228_DT_dac2_mixer_mode "Mixer Mode"; t228_DT_dac2_nco_freq "NCO Frequency (GHz)"; t228_DT_dac2_nco_phase "NCO Phase"; t228_DT_dac2_coarse_freq "Frequency"; t228_DT_dac2_nyquist_zone "Nyquist Zone"; t228_DT_dac2_decode_mode "Decoder Mode"; t228_DT_dac3_enable "Enable DAC"; t228_DT_dac3_analog_output "Analog Output Data"; t228_DT_dac3_inter_mode "Interpolation Mode"; t228_DT_dac3_sample_per_cycle "Samples per AXI4-Stream Cycle"; t228_DT_dac3_mixer_type "Mixer Type"; t228_DT_dac3_mixer_mode "Mixer Mode"; t228_DT_dac3_nco_freq "NCO Frequency (GHz)"; t228_DT_dac3_nco_phase "NCO Phase"; t228_DT_dac3_coarse_freq "Frequency"; t228_DT_dac3_nyquist_zone "Nyquist Zone"; t228_DT_dac3_decode_mode "Decoder Mode"; Tile229_enable "Enable Tile"; t229_enable_mts "Enable Multi-Tile Sync"; t229_sample_rate "Sampling Rate (Msps)"; t229_clk_out "Clock Out (MHz)"; t229_enable_pll "Enable Tile PLLs"; t229_ref_clk "Reference Clock (MHz)"; t229_axi_stream_clk "Required AXI4-Stream Clock (MHz)"; t229_output_power "Output Power"; t229_QT_dac0_enable "Enable DAC"; t229_QT_dac0_analog_output "Analog Output Data"; t229_QT_dac0_inter_mode "Interpolation Mode"; t229_QT_dac0_sample_per_cycle "Samples per AXI4-Stream Cycle"; t229_QT_dac0_datapath_mode "Datapath Mode"; t229_QT_dac0_mixer_type "Mixer Type"; t229_QT_dac0_mixer_mode "Mixer Mode"; t229_QT_dac0_nco_freq "NCO Frequency (GHz)"; t229_QT_dac0_nco_phase "NCO Phase"; t229_QT_dac0_coarse_freq "Frequency"; t229_QT_dac0_nyquist_zone "Nyquist Zone"; t229_QT_dac0_decode_mode "Decoder Mode"; t229_QT_dac1_enable "Enable DAC"; t229_QT_dac1_analog_output "Analog Output Data"; t229_QT_dac1_inter_mode "Interpolation Mode"; t229_QT_dac1_sample_per_cycle "Samples per AXI4-Stream Cycle"; t229_QT_dac1_datapath_mode "Datapath Mode"; t229_QT_dac1_mixer_type "Mixer Type"; t229_QT_dac1_mixer_mode "Mixer Mode"; t229_QT_dac1_nco_freq "NCO Frequency (GHz)"; t229_QT_dac1_nco_phase "NCO Phase"; t229_QT_dac1_coarse_freq "Frequency"; t229_QT_dac1_nyquist_zone "Nyquist Zone"; t229_QT_dac1_decode_mode "Decoder Mode"; t229_QT_dac2_enable "Enable DAC"; t229_QT_dac2_analog_output "Analog Output Data"; t229_QT_dac2_inter_mode "Interpolation Mode"; t229_QT_dac2_sample_per_cycle "Samples per AXI4-Stream Cycle"; t229_QT_dac2_datapath_mode "Datapath Mode"; t229_QT_dac2_mixer_type "Mixer Type"; t229_QT_dac2_mixer_mode "Mixer Mode"; t229_QT_dac2_nco_freq "NCO Frequency (GHz)"; t229_QT_dac2_nco_phase "NCO Phase"; t229_QT_dac2_coarse_freq "Frequency"; t229_QT_dac2_nyquist_zone "Nyquist Zone"; t229_QT_dac2_decode_mode "Decoder Mode"; t229_QT_dac3_enable "Enable DAC"; t229_QT_dac3_analog_output "Analog Output Data"; t229_QT_dac3_inter_mode "Interpolation Mode"; t229_QT_dac3_sample_per_cycle "Samples per AXI4-Stream Cycle"; t229_QT_dac3_datapath_mode "Datapath Mode"; t229_QT_dac3_mixer_type "Mixer Type"; t229_QT_dac3_mixer_mode "Mixer Mode"; t229_QT_dac3_nco_freq "NCO Frequency (GHz)"; t229_QT_dac3_nco_phase "NCO Phase"; t229_QT_dac3_coarse_freq "Frequency"; t229_QT_dac3_nyquist_zone "Nyquist Zone"; t229_QT_dac3_decode_mode "Decoder Mode"; t229_DT_dac0_enable "Enable DAC"; t229_DT_dac0_analog_output "Analog Output Data"; t229_DT_dac0_inter_mode "Interpolation Mode"; t229_DT_dac0_sample_per_cycle "Samples per AXI4-Stream Cycle"; t229_DT_dac0_mixer_type "Mixer Type"; t229_DT_dac0_mixer_mode "Mixer Mode"; t229_DT_dac0_nco_freq "NCO Frequency (GHz)"; t229_DT_dac0_nco_phase "NCO Phase"; t229_DT_dac0_coarse_freq "Frequency"; t229_DT_dac0_nyquist_zone "Nyquist Zone"; t229_DT_dac0_decode_mode "Decoder Mode"; t229_DT_dac1_enable "Enable DAC"; t229_DT_dac1_analog_output "Analog Output Data"; t229_DT_dac1_inter_mode "Interpolation Mode"; t229_DT_dac1_sample_per_cycle "Samples per AXI4-Stream Cycle"; t229_DT_dac1_mixer_type "Mixer Type"; t229_DT_dac1_mixer_mode "Mixer Mode"; t229_DT_dac1_nco_freq "NCO Frequency (GHz)"; t229_DT_dac1_nco_phase "NCO Phase"; t229_DT_dac1_coarse_freq "Frequency"; t229_DT_dac1_nyquist_zone "Nyquist Zone"; t229_DT_dac1_decode_mode "Decoder Mode"; t229_DT_dac2_enable "Enable DAC"; t229_DT_dac2_analog_output "Analog Output Data"; t229_DT_dac2_inter_mode "Interpolation Mode"; t229_DT_dac2_sample_per_cycle "Samples per AXI4-Stream Cycle"; t229_DT_dac2_mixer_type "Mixer Type"; t229_DT_dac2_mixer_mode "Mixer Mode"; t229_DT_dac2_nco_freq "NCO Frequency (GHz)"; t229_DT_dac2_nco_phase "NCO Phase"; t229_DT_dac2_coarse_freq "Frequency"; t229_DT_dac2_nyquist_zone "Nyquist Zone"; t229_DT_dac2_decode_mode "Decoder Mode"; t229_DT_dac3_enable "Enable DAC"; t229_DT_dac3_analog_output "Analog Output Data"; t229_DT_dac3_inter_mode "Interpolation Mode"; t229_DT_dac3_sample_per_cycle "Samples per AXI4-Stream Cycle"; t229_DT_dac3_mixer_type "Mixer Type"; t229_DT_dac3_mixer_mode "Mixer Mode"; t229_DT_dac3_nco_freq "NCO Frequency (GHz)"; t229_DT_dac3_nco_phase "NCO Phase"; t229_DT_dac3_coarse_freq "Frequency"; t229_DT_dac3_nyquist_zone "Nyquist Zone"; t229_DT_dac3_decode_mode "Decoder Mode"; Tile230_enable "Enable Tile"; t230_enable_mts "Enable Multi-Tile Sync"; t230_sample_rate "Sampling Rate (Msps)"; t230_clk_out "Clock Out (MHz)"; t230_enable_pll "Enable Tile PLLs"; t230_ref_clk "Reference Clock (MHz)"; t230_axi_stream_clk "Required AXI4-Stream Clock (MHz)"; t230_output_power "Output Power"; t230_QT_dac0_enable "Enable DAC"; t230_QT_dac0_analog_output "Analog Output Data"; t230_QT_dac0_inter_mode "Interpolation Mode"; t230_QT_dac0_sample_per_cycle "Samples per AXI4-Stream Cycle"; t230_QT_dac0_datapath_mode "Datapath Mode"; t230_QT_dac0_mixer_type "Mixer Type"; t230_QT_dac0_mixer_mode "Mixer Mode"; t230_QT_dac0_nco_freq "NCO Frequency (GHz)"; t230_QT_dac0_nco_phase "NCO Phase"; t230_QT_dac0_coarse_freq "Frequency"; t230_QT_dac0_nyquist_zone "Nyquist Zone"; t230_QT_dac0_decode_mode "Decoder Mode"; t230_QT_dac1_enable "Enable DAC"; t230_QT_dac1_analog_output "Analog Output Data"; t230_QT_dac1_inter_mode "Interpolation Mode"; t230_QT_dac1_sample_per_cycle "Samples per AXI4-Stream Cycle"; t230_QT_dac1_datapath_mode "Datapath Mode"; t230_QT_dac1_mixer_type "Mixer Type"; t230_QT_dac1_mixer_mode "Mixer Mode"; t230_QT_dac1_nco_freq "NCO Frequency (GHz)"; t230_QT_dac1_nco_phase "NCO Phase"; t230_QT_dac1_coarse_freq "Frequency"; t230_QT_dac1_nyquist_zone "Nyquist Zone"; t230_QT_dac1_decode_mode "Decoder Mode"; t230_QT_dac2_enable "Enable DAC"; t230_QT_dac2_analog_output "Analog Output Data"; t230_QT_dac2_inter_mode "Interpolation Mode"; t230_QT_dac2_sample_per_cycle "Samples per AXI4-Stream Cycle"; t230_QT_dac2_datapath_mode "Datapath Mode"; t230_QT_dac2_mixer_type "Mixer Type"; t230_QT_dac2_mixer_mode "Mixer Mode"; t230_QT_dac2_nco_freq "NCO Frequency (GHz)"; t230_QT_dac2_nco_phase "NCO Phase"; t230_QT_dac2_coarse_freq "Frequency"; t230_QT_dac2_nyquist_zone "Nyquist Zone"; t230_QT_dac2_decode_mode "Decoder Mode"; t230_QT_dac3_enable "Enable DAC"; t230_QT_dac3_analog_output "Analog Output Data"; t230_QT_dac3_inter_mode "Interpolation Mode"; t230_QT_dac3_sample_per_cycle "Samples per AXI4-Stream Cycle"; t230_QT_dac3_datapath_mode "Datapath Mode"; t230_QT_dac3_mixer_type "Mixer Type"; t230_QT_dac3_mixer_mode "Mixer Mode"; t230_QT_dac3_nco_freq "NCO Frequency (GHz)"; t230_QT_dac3_nco_phase "NCO Phase"; t230_QT_dac3_coarse_freq "Frequency"; t230_QT_dac3_nyquist_zone "Nyquist Zone"; t230_QT_dac3_decode_mode "Decoder Mode"; Tile231_enable "Enable Tile"; t231_enable_mts "Enable Multi-Tile Sync"; t231_sample_rate "Sampling Rate (Msps)"; t231_clk_out "Clock Out (MHz)"; t231_enable_pll "Enable Tile PLLs"; t231_ref_clk "Reference Clock (MHz)"; t231_axi_stream_clk "Required AXI4-Stream Clock (MHz)"; t231_output_power "Output Power"; t231_QT_dac0_enable "Enable DAC"; t231_QT_dac0_analog_output "Analog Output Data"; t231_QT_dac0_inter_mode "Interpolation Mode"; t231_QT_dac0_sample_per_cycle "Samples per AXI4-Stream Cycle"; t231_QT_dac0_datapath_mode "Datapath Mode"; t231_QT_dac0_mixer_type "Mixer Type"; t231_QT_dac0_mixer_mode "Mixer Mode"; t231_QT_dac0_nco_freq "NCO Frequency (GHz)"; t231_QT_dac0_nco_phase "NCO Phase"; t231_QT_dac0_coarse_freq "Frequency"; t231_QT_dac0_nyquist_zone "Nyquist Zone"; t231_QT_dac0_decode_mode "Decoder Mode"; t231_QT_dac1_enable "Enable DAC"; t231_QT_dac1_analog_output "Analog Output Data"; t231_QT_dac1_inter_mode "Interpolation Mode"; t231_QT_dac1_sample_per_cycle "Samples per AXI4-Stream Cycle"; t231_QT_dac1_datapath_mode "Datapath Mode"; t231_QT_dac1_mixer_type "Mixer Type"; t231_QT_dac1_mixer_mode "Mixer Mode"; t231_QT_dac1_nco_freq "NCO Frequency (GHz)"; t231_QT_dac1_nco_phase "NCO Phase"; t231_QT_dac1_coarse_freq "Frequency"; t231_QT_dac1_nyquist_zone "Nyquist Zone"; t231_QT_dac1_decode_mode "Decoder Mode"; t231_QT_dac2_enable "Enable DAC"; t231_QT_dac2_analog_output "Analog Output Data"; t231_QT_dac2_inter_mode "Interpolation Mode"; t231_QT_dac2_sample_per_cycle "Samples per AXI4-Stream Cycle"; t231_QT_dac2_datapath_mode "Datapath Mode"; t231_QT_dac2_mixer_type "Mixer Type"; t231_QT_dac2_mixer_mode "Mixer Mode"; t231_QT_dac2_nco_freq "NCO Frequency (GHz)"; t231_QT_dac2_nco_phase "NCO Phase"; t231_QT_dac2_coarse_freq "Frequency"; t231_QT_dac2_nyquist_zone "Nyquist Zone"; t231_QT_dac2_decode_mode "Decoder Mode"; t231_QT_dac3_enable "Enable DAC"; t231_QT_dac3_analog_output "Analog Output Data"; t231_QT_dac3_inter_mode "Interpolation Mode"; t231_QT_dac3_sample_per_cycle "Samples per AXI4-Stream Cycle"; t231_QT_dac3_datapath_mode "Datapath Mode"; t231_QT_dac3_mixer_type "Mixer Type"; t231_QT_dac3_mixer_mode "Mixer Mode"; t231_QT_dac3_nco_freq "NCO Frequency (GHz)"; t231_QT_dac3_nco_phase "NCO Phase"; t231_QT_dac3_coarse_freq "Frequency"; t231_QT_dac3_nyquist_zone "Nyquist Zone"; t231_QT_dac3_decode_mode "Decoder Mode"; t224_has_adc_clk "Has Clock"; t224_adc_clk_src "Clock Source Tile"; t224_clk_dist "Distribute Clock"; t225_has_adc_clk "Has Clock"; t225_adc_clk_src "Clock Source Tile"; t225_clk_dist "Distribute Clock"; t226_has_adc_clk "Has Clock"; t226_adc_clk_src "Clock Source Tile"; t226_clk_dist "Distribute Clock"; t227_has_adc_clk "Has Clock"; t227_adc_clk_src "Clock Source Tile"; t227_clk_dist "Distribute Clock"; t228_has_dac_clk "Has Clock"; t228_dac_clk_src "Clock Source Tile"; t228_clk_dist "Distribute Clock"; t229_has_dac_clk "Has Clock"; t229_dac_clk_src "Clock Source Tile"; t229_clk_dist "Distribute Clock"; t230_has_dac_clk "Has Clock"; t230_dac_clk_src "Clock Source Tile"; t230_clk_dist "Distribute Clock"; t231_has_dac_clk "Has Clock"; t231_dac_clk_src "Clock Source Tile"; t231_clk_dist "Distribute Clock"
      mask help: CASPER RFDC
      mask init:
      | if chk_param(gcb,'runinit','1')
      |     if chk_param(gcb,'forceredraw','0')
      |         rfdc_mask(gcb,0);
      |     else
      |         rfdc_mask(gcb,1);
      |         set_param(gcb,'forceredraw','0')
      |     end
      |     if chk_param(gcb,'maskopening','1')
      |         set_param(gcb,'runinit','0')
      |   end
      | end
      mask Help: eval('xlWeb([getenv(''MLIB_ROOT''), ''\doc\html\adc_zcu111\adc_zcu111.html''])')
      mask Callback maskopening:
      | %assignin('base','mask_opening',1)
      | %assignin('base','run_init',1)
      | set_param(gcb,'maskopening','1')
      mask Callback runinit: set_param(gcb,'runinit','1')
      mask Callback Tile224_enable: enable_mts_opt(gcb);
      mask Callback t224_sample_rate: update_rfdc_clocking(gcb,224);
      mask TypeOptions t224_clk_out: 125 | 62.5 | 31.25 | 15.625
      mask Callback t224_enable_pll:
      | %update_rfdc_clocking(gcb);
      | update_pll(gcb,224);
      mask TypeOptions t224_ref_clk: 923.077 | 857.143 | 800 | 750 | 705.882 | 666.667 | 631.579 | 600 | 571.429 | 545.455 | 521.739 | 500 | 480 | 461.538 | 444.444 | 428.571 | 413.793 | 400 | 387.097 | 375 | 363.636 | 352.941 | 342.857 | 333.333 | 324.324 | 315.789 | 307.692 | 300 | 292.683 | 285.714 | 279.07 | 272.727 | 266.667 | 260.87 | 255.319 | 250 | 244.898 | 240 | 235.294 | 230.769 | 226.415 | 222.222 | 218.182 | 214.286 | 210.526 | 206.897 | 203.39 | 200 | 196.721 | 193.548 | 190.476 | 187.5 | 184.615 | 181.818 | 179.104 | 176.471 | 173.913 | 171.429 | 169.014 | 166.667 | 164.384 | 162.162 | 160 | 157.895 | 155.844 | 153.846 | 151.899 | 150 | 148.148 | 146.341 | 144.578 | 142.857 | 141.176 | 139.535 | 137.931 | 136.364 | 134.831 | 133.333 | 131.868 | 130.435 | 129.032 | 127.66 | 126.316 | 125 | 123.711 | 122.449 | 121.212 | 120 | 118.812 | 117.647 | 116.505 | 115.385 | 114.286 | 113.208 | 112.15 | 111.111 | 110.092 | 109.091 | 108.108 | 107.143 | 106.195 | 105.263 | 104.348 | 103.448 | 102.564
      mask Callback t224_QT_adc0_enable: enable_adc_opt(gcb,224,0);
      mask TypeOptions t224_QT_adc0_digital_output: Real | I/Q
      mask Callback t224_QT_adc0_digital_output:
      | validate_digital_data(gcb,224,0,'QT');
      | update_axis_clk(gcb,224);
      mask TypeOptions t224_QT_adc0_dec_mode: 1x | 2x | 4x | 8x
      mask Callback t224_QT_adc0_dec_mode: update_axis_clk(gcb,224);
      mask TypeOptions t224_QT_adc0_sample_per_cycle: 2 | 4 | 6 | 8 | 10 | 12
      mask Callback t224_QT_adc0_sample_per_cycle:
      | %update_axis_clk(gcb);
      | update_axis_clk_label(gcb,224);
      mask TypeOptions t224_QT_adc0_mixer_type: Fine | Coarse
      mask Callback t224_QT_adc0_mixer_type: mixertype_callback(gcb,224,0,'QT');
      mask TypeOptions t224_QT_adc0_mixer_mode: Real -> I/Q | I/Q -> I/Q
      mask Callback t224_QT_adc0_mixer_mode: mixer_callback(gcb,224,0,'QT');
      mask TypeOptions t224_QT_adc0_coarse_freq: 0
      mask TypeOptions t224_QT_adc0_nyquist_zone: Zone 1 | Zone 2
      mask TypeOptions t224_QT_adc0_cal_mode: Mode 1 | Mode 2
      mask Callback t224_QT_adc1_enable: enable_adc_opt(gcb,224,1);
      mask TypeOptions t224_QT_adc1_digital_output: Real | I/Q
      mask Callback t224_QT_adc1_digital_output:
      | validate_digital_data(gcb,224,1,'QT');
      | update_axis_clk(gcb,224);
      mask TypeOptions t224_QT_adc1_dec_mode: 1x | 2x | 4x | 8x
      mask Callback t224_QT_adc1_dec_mode: update_axis_clk(gcb,224);
      mask TypeOptions t224_QT_adc1_sample_per_cycle: 2 | 4 | 6 | 8 | 10 | 12
      mask Callback t224_QT_adc1_sample_per_cycle: update_axis_clk_label(gcb,224);
      mask TypeOptions t224_QT_adc1_mixer_type: Fine | Coarse
      mask Callback t224_QT_adc1_mixer_type: mixertype_callback(gcb,224,1,'QT');
      mask TypeOptions t224_QT_adc1_mixer_mode: Real -> I/Q
      mask Callback t224_QT_adc1_mixer_mode: mixer_callback(gcb,224,1,'QT')
      mask TypeOptions t224_QT_adc1_coarse_freq: 0
      mask TypeOptions t224_QT_adc1_nyquist_zone: Zone 1 | Zone 2
      mask TypeOptions t224_QT_adc1_cal_mode: Mode 1 | Mode 2
      mask Callback t224_QT_adc2_enable: enable_adc_opt(gcb,224,2);
      mask TypeOptions t224_QT_adc2_digital_output: Real | I/Q
      mask Callback t224_QT_adc2_digital_output:
      | validate_digital_data(gcb,224,2,'QT');
      | update_axis_clk(gcb,224);
      mask TypeOptions t224_QT_adc2_dec_mode: 1x | 2x | 4x | 8x
      mask Callback t224_QT_adc2_dec_mode: update_axis_clk(gcb,224);
      mask TypeOptions t224_QT_adc2_sample_per_cycle: 2 | 4 | 6 | 8 | 10 | 12
      mask Callback t224_QT_adc2_sample_per_cycle: update_axis_clk_label(gcb,224);
      mask TypeOptions t224_QT_adc2_mixer_type: Fine | Coarse
      mask Callback t224_QT_adc2_mixer_type: mixertype_callback(gcb,224,2,'QT');
      mask TypeOptions t224_QT_adc2_mixer_mode: Real -> I/Q | I/Q -> I/Q
      mask Callback t224_QT_adc2_mixer_mode: mixer_callback(gcb,224,2,'QT')
      mask TypeOptions t224_QT_adc2_coarse_freq: 0
      mask TypeOptions t224_QT_adc2_nyquist_zone: Zone 1 | Zone 2
      mask TypeOptions t224_QT_adc2_cal_mode: Mode 1 | Mode 2
      mask Callback t224_QT_adc3_enable: enable_adc_opt(gcb,224,3);
      mask TypeOptions t224_QT_adc3_digital_output: Real | I/Q
      mask Callback t224_QT_adc3_digital_output:
      | validate_digital_data(gcb,224,3,'QT');
      | update_axis_clk(gcb,224);
      mask TypeOptions t224_QT_adc3_dec_mode: 1x | 2x | 4x | 8x
      mask Callback t224_QT_adc3_dec_mode: update_axis_clk(gcb,224);
      mask TypeOptions t224_QT_adc3_sample_per_cycle: 2 | 4 | 6 | 8 | 10 | 12
      mask Callback t224_QT_adc3_sample_per_cycle: update_axis_clk_label(gcb,224);
      mask TypeOptions t224_QT_adc3_mixer_type: Fine | Coarse
      mask Callback t224_QT_adc3_mixer_type: mixertype_callback(gcb,224,3,'QT');
      mask TypeOptions t224_QT_adc3_mixer_mode: Real -> I/Q
      mask Callback t224_QT_adc3_mixer_mode: mixer_callback(gcb,224,3,'QT')
      mask TypeOptions t224_QT_adc3_coarse_freq: 0
      mask TypeOptions t224_QT_adc3_nyquist_zone: Zone 1 | Zone 2
      mask TypeOptions t224_QT_adc3_cal_mode: Mode 1 | Mode 2
      mask Callback t224_DT_adc0_enable: enable_adc_opt(gcb,224,0);
      mask TypeOptions t224_DT_adc0_digital_output: Real | I/Q
      mask Callback t224_DT_adc0_digital_output:
      | validate_digital_data(gcb,224,0,'DT');
      | update_axis_clk(gcb,224);
      mask TypeOptions t224_DT_adc0_dec_mode: 1x | 2x | 4x | 8x
      mask Callback t224_DT_adc0_dec_mode: update_axis_clk(gcb,224);
      mask TypeOptions t224_DT_adc0_sample_per_cycle: 2 | 3 | 4 | 5 | 6 | 7 | 8
      mask Callback t224_DT_adc0_sample_per_cycle:
      | %update_axis_clk(gcb);
      | update_axis_clk_label(gcb,224);
      mask TypeOptions t224_DT_adc0_mixer_type: Bypassed
      mask Callback t224_DT_adc0_mixer_type: mixertype_callback(gcb,224,0,'DT');
      mask TypeOptions t224_DT_adc0_mixer_mode: Real -> Real
      mask Callback t224_DT_adc0_mixer_mode: mixer_callback(gcb,224,0,'DT');
      mask TypeOptions t224_DT_adc0_coarse_freq: 0
      mask TypeOptions t224_DT_adc0_nyquist_zone: Zone 1 | Zone 2
      mask TypeOptions t224_DT_adc0_cal_mode: Mode 1 | Mode 2
      mask Callback t224_DT_adc1_enable: enable_adc_opt(gcb,224,1);
      mask TypeOptions t224_DT_adc1_digital_output: Real | I/Q
      mask Callback t224_DT_adc1_digital_output:
      | validate_digital_data(gcb,224,1,'DT');
      | update_axis_clk(gcb,224);
      mask TypeOptions t224_DT_adc1_dec_mode: 1x | 2x | 4x | 8x
      mask Callback t224_DT_adc1_dec_mode: update_axis_clk(gcb,224);
      mask TypeOptions t224_DT_adc1_sample_per_cycle: 2 | 3 | 4 | 5 | 6 | 7 | 8
      mask Callback t224_DT_adc1_sample_per_cycle:
      | %update_axis_clk(gcb);
      | update_axis_clk_label(gcb,224);
      mask TypeOptions t224_DT_adc1_mixer_type: Bypassed
      mask Callback t224_DT_adc1_mixer_type: mixertype_callback(gcb,224,1,'DT');
      mask TypeOptions t224_DT_adc1_mixer_mode: Real -> Real
      mask Callback t224_DT_adc1_mixer_mode: mixer_callback(gcb,224,1,'DT');
      mask TypeOptions t224_DT_adc1_coarse_freq: 0
      mask TypeOptions t224_DT_adc1_nyquist_zone: Zone 1 | Zone 2
      mask TypeOptions t224_DT_adc1_cal_mode: Mode 1 | Mode 2
      mask Callback t225_sample_rate: update_rfdc_clocking(gcb,225);
      mask TypeOptions t225_clk_out: 125 | 62.5 | 31.25 | 15.625
      mask Callback t225_enable_pll:
      | %update_rfdc_clocking(gcb);
      | update_pll(gcb,225);
      mask TypeOptions t225_ref_clk: 923.077 | 857.143 | 800 | 750 | 705.882 | 666.667 | 631.579 | 600 | 571.429 | 545.455 | 521.739 | 500 | 480 | 461.538 | 444.444 | 428.571 | 413.793 | 400 | 387.097 | 375 | 363.636 | 352.941 | 342.857 | 333.333 | 324.324 | 315.789 | 307.692 | 300 | 292.683 | 285.714 | 279.07 | 272.727 | 266.667 | 260.87 | 255.319 | 250 | 244.898 | 240 | 235.294 | 230.769 | 226.415 | 222.222 | 218.182 | 214.286 | 210.526 | 206.897 | 203.39 | 200 | 196.721 | 193.548 | 190.476 | 187.5 | 184.615 | 181.818 | 179.104 | 176.471 | 173.913 | 171.429 | 169.014 | 166.667 | 164.384 | 162.162 | 160 | 157.895 | 155.844 | 153.846 | 151.899 | 150 | 148.148 | 146.341 | 144.578 | 142.857 | 141.176 | 139.535 | 137.931 | 136.364 | 134.831 | 133.333 | 131.868 | 130.435 | 129.032 | 127.66 | 126.316 | 125 | 123.711 | 122.449 | 121.212 | 120 | 118.812 | 117.647 | 116.505 | 115.385 | 114.286 | 113.208 | 112.15 | 111.111 | 110.092 | 109.091 | 108.108 | 107.143 | 106.195 | 105.263 | 104.348 | 103.448 | 102.564
      mask Callback t225_QT_adc0_enable: enable_adc_opt(gcb,225,0);
      mask TypeOptions t225_QT_adc0_digital_output: Real | I/Q
      mask Callback t225_QT_adc0_digital_output:
      | validate_digital_data(gcb,225,0,'QT');
      | update_axis_clk(gcb,225);
      mask TypeOptions t225_QT_adc0_dec_mode: 1x | 2x | 4x | 8x
      mask Callback t225_QT_adc0_dec_mode: update_axis_clk(gcb,225);
      mask TypeOptions t225_QT_adc0_sample_per_cycle: 1 | 2 | 3 | 4 | 5 | 6 | 7 | 8 | 9 | 10 | 11 | 12
      mask Callback t225_QT_adc0_sample_per_cycle:
      | %update_axis_clk(gcb);
      | update_axis_clk_label(gcb,225);
      mask TypeOptions t225_QT_adc0_mixer_type: Bypassed
      mask Callback t225_QT_adc0_mixer_type: mixertype_callback(gcb,225,0,'QT');
      mask TypeOptions t225_QT_adc0_mixer_mode: Real -> Real
      mask Callback t225_QT_adc0_mixer_mode: mixer_callback(gcb,225,0,'QT');
      mask TypeOptions t225_QT_adc0_coarse_freq: 0
      mask TypeOptions t225_QT_adc0_nyquist_zone: Zone 1 | Zone 2
      mask TypeOptions t225_QT_adc0_cal_mode: Mode 1 | Mode 2
      mask Callback t225_QT_adc1_enable: enable_adc_opt(gcb,225,1);
      mask TypeOptions t225_QT_adc1_digital_output: Real | I/Q
      mask Callback t225_QT_adc1_digital_output:
      | validate_digital_data(gcb,225,1,'QT');
      | update_axis_clk(gcb,225);
      mask TypeOptions t225_QT_adc1_dec_mode: 1x | 2x | 4x | 8x
      mask Callback t225_QT_adc1_dec_mode: update_axis_clk(gcb,225);
      mask TypeOptions t225_QT_adc1_sample_per_cycle: 1 | 2 | 3 | 4 | 5 | 6 | 7 | 8 | 9 | 10 | 11 | 12
      mask Callback t225_QT_adc1_sample_per_cycle: update_axis_clk_label(gcb,225);
      mask TypeOptions t225_QT_adc1_mixer_type: Bypassed
      mask Callback t225_QT_adc1_mixer_type: mixertype_callback(gcb,225,1,'QT');
      mask TypeOptions t225_QT_adc1_mixer_mode: Real -> Real
      mask Callback t225_QT_adc1_mixer_mode: mixer_callback(gcb,225,1,'QT')
      mask TypeOptions t225_QT_adc1_coarse_freq: 0
      mask TypeOptions t225_QT_adc1_nyquist_zone: Zone 1 | Zone 2
      mask TypeOptions t225_QT_adc1_cal_mode: Mode 1 | Mode 2
      mask Callback t225_QT_adc2_enable: enable_adc_opt(gcb,225,2);
      mask TypeOptions t225_QT_adc2_digital_output: Real | I/Q
      mask Callback t225_QT_adc2_digital_output:
      | validate_digital_data(gcb,225,2,'QT');
      | update_axis_clk(gcb,225);
      mask TypeOptions t225_QT_adc2_dec_mode: 1x | 2x | 4x | 8x
      mask Callback t225_QT_adc2_dec_mode: update_axis_clk(gcb,225);
      mask TypeOptions t225_QT_adc2_sample_per_cycle: 1 | 2 | 3 | 4 | 5 | 6 | 7 | 8 | 9 | 10 | 11 | 12
      mask Callback t225_QT_adc2_sample_per_cycle: update_axis_clk_label(gcb,225);
      mask TypeOptions t225_QT_adc2_mixer_type: Bypassed
      mask Callback t225_QT_adc2_mixer_type: mixertype_callback(gcb,225,2,'QT');
      mask TypeOptions t225_QT_adc2_mixer_mode: Real -> Real
      mask Callback t225_QT_adc2_mixer_mode: mixer_callback(gcb,225,2,'QT')
      mask TypeOptions t225_QT_adc2_coarse_freq: 0
      mask TypeOptions t225_QT_adc2_nyquist_zone: Zone 1 | Zone 2
      mask TypeOptions t225_QT_adc2_cal_mode: Mode 1 | Mode 2
      mask Callback t225_QT_adc3_enable: enable_adc_opt(gcb,225,3);
      mask TypeOptions t225_QT_adc3_digital_output: Real | I/Q
      mask Callback t225_QT_adc3_digital_output:
      | validate_digital_data(gcb,225,3,'QT');
      | update_axis_clk(gcb,225);
      mask TypeOptions t225_QT_adc3_dec_mode: 1x | 2x | 4x | 8x
      mask Callback t225_QT_adc3_dec_mode: update_axis_clk(gcb,225);
      mask TypeOptions t225_QT_adc3_sample_per_cycle: 1 | 2 | 3 | 4 | 5 | 6 | 7 | 8 | 9 | 10 | 11 | 12
      mask Callback t225_QT_adc3_sample_per_cycle: update_axis_clk_label(gcb,225);
      mask TypeOptions t225_QT_adc3_mixer_type: Bypassed
      mask Callback t225_QT_adc3_mixer_type: mixertype_callback(gcb,225,3,'QT');
      mask TypeOptions t225_QT_adc3_mixer_mode: Real -> Real
      mask Callback t225_QT_adc3_mixer_mode: mixer_callback(gcb,225,3,'QT')
      mask TypeOptions t225_QT_adc3_coarse_freq: 0
      mask TypeOptions t225_QT_adc3_nyquist_zone: Zone 1 | Zone 2
      mask TypeOptions t225_QT_adc3_cal_mode: Mode 1 | Mode 2
      mask Callback t225_DT_adc0_enable: enable_adc_opt(gcb,225,0);
      mask TypeOptions t225_DT_adc0_digital_output: Real | I/Q
      mask Callback t225_DT_adc0_digital_output:
      | validate_digital_data(gcb,225,0,'DT');
      | update_axis_clk(gcb,225);
      mask TypeOptions t225_DT_adc0_dec_mode: 1x | 2x | 4x | 8x
      mask Callback t225_DT_adc0_dec_mode: update_axis_clk(gcb,225);
      mask TypeOptions t225_DT_adc0_sample_per_cycle: 2 | 3 | 4 | 5 | 6 | 7 | 8
      mask Callback t225_DT_adc0_sample_per_cycle:
      | %update_axis_clk(gcb);
      | update_axis_clk_label(gcb,225);
      mask TypeOptions t225_DT_adc0_mixer_type: Bypassed
      mask Callback t225_DT_adc0_mixer_type: mixertype_callback(gcb,225,0,'DT');
      mask TypeOptions t225_DT_adc0_mixer_mode: Real -> Real
      mask Callback t225_DT_adc0_mixer_mode: mixer_callback(gcb,225,0,'DT');
      mask TypeOptions t225_DT_adc0_coarse_freq: 0
      mask TypeOptions t225_DT_adc0_nyquist_zone: Zone 1 | Zone 2
      mask TypeOptions t225_DT_adc0_cal_mode: Mode 1 | Mode 2
      mask Callback t225_DT_adc1_enable: enable_adc_opt(gcb,225,1);
      mask TypeOptions t225_DT_adc1_digital_output: Real | I/Q
      mask Callback t225_DT_adc1_digital_output:
      | validate_digital_data(gcb,225,1,'DT');
      | update_axis_clk(gcb,225);
      mask TypeOptions t225_DT_adc1_dec_mode: 1x | 2x | 4x | 8x
      mask Callback t225_DT_adc1_dec_mode: update_axis_clk(gcb,225);
      mask TypeOptions t225_DT_adc1_sample_per_cycle: 2 | 3 | 4 | 5 | 6 | 7 | 8
      mask Callback t225_DT_adc1_sample_per_cycle:
      | %update_axis_clk(gcb);
      | update_axis_clk_label(gcb,225);
      mask TypeOptions t225_DT_adc1_mixer_type: Bypassed
      mask Callback t225_DT_adc1_mixer_type: mixertype_callback(gcb,225,1,'DT');
      mask TypeOptions t225_DT_adc1_mixer_mode: Real -> Real
      mask Callback t225_DT_adc1_mixer_mode: mixer_callback(gcb,225,1,'DT');
      mask TypeOptions t225_DT_adc1_coarse_freq: 0
      mask TypeOptions t225_DT_adc1_nyquist_zone: Zone 1 | Zone 2
      mask TypeOptions t225_DT_adc1_cal_mode: Mode 1 | Mode 2
      mask Callback t226_sample_rate: update_rfdc_clocking(gcb,226);
      mask TypeOptions t226_clk_out: 125 | 62.5 | 31.25 | 15.625
      mask Callback t226_enable_pll:
      | %update_rfdc_clocking(gcb);
      | update_pll(gcb,226);
      mask TypeOptions t226_ref_clk: 923.077 | 857.143 | 800 | 750 | 705.882 | 666.667 | 631.579 | 600 | 571.429 | 545.455 | 521.739 | 500 | 480 | 461.538 | 444.444 | 428.571 | 413.793 | 400 | 387.097 | 375 | 363.636 | 352.941 | 342.857 | 333.333 | 324.324 | 315.789 | 307.692 | 300 | 292.683 | 285.714 | 279.07 | 272.727 | 266.667 | 260.87 | 255.319 | 250 | 244.898 | 240 | 235.294 | 230.769 | 226.415 | 222.222 | 218.182 | 214.286 | 210.526 | 206.897 | 203.39 | 200 | 196.721 | 193.548 | 190.476 | 187.5 | 184.615 | 181.818 | 179.104 | 176.471 | 173.913 | 171.429 | 169.014 | 166.667 | 164.384 | 162.162 | 160 | 157.895 | 155.844 | 153.846 | 151.899 | 150 | 148.148 | 146.341 | 144.578 | 142.857 | 141.176 | 139.535 | 137.931 | 136.364 | 134.831 | 133.333 | 131.868 | 130.435 | 129.032 | 127.66 | 126.316 | 125 | 123.711 | 122.449 | 121.212 | 120 | 118.812 | 117.647 | 116.505 | 115.385 | 114.286 | 113.208 | 112.15 | 111.111 | 110.092 | 109.091 | 108.108 | 107.143 | 106.195 | 105.263 | 104.348 | 103.448 | 102.564
      mask Callback t226_QT_adc0_enable: enable_adc_opt(gcb,226,0);
      mask TypeOptions t226_QT_adc0_digital_output: Real | I/Q
      mask Callback t226_QT_adc0_digital_output:
      | validate_digital_data(gcb,226,0,'QT');
      | update_axis_clk(gcb,226);
      mask TypeOptions t226_QT_adc0_dec_mode: 1x | 2x | 4x | 8x
      mask Callback t226_QT_adc0_dec_mode: update_axis_clk(gcb,226);
      mask TypeOptions t226_QT_adc0_sample_per_cycle: 1 | 2 | 3 | 4 | 5 | 6 | 7 | 8 | 9 | 10 | 11 | 12
      mask Callback t226_QT_adc0_sample_per_cycle:
      | %update_axis_clk(gcb);
      | update_axis_clk_label(gcb,226);
      mask TypeOptions t226_QT_adc0_mixer_type: Bypassed
      mask Callback t226_QT_adc0_mixer_type: mixertype_callback(gcb,226,0,'QT');
      mask TypeOptions t226_QT_adc0_mixer_mode: Real -> Real
      mask Callback t226_QT_adc0_mixer_mode: mixer_callback(gcb,226,0,'QT');
      mask TypeOptions t226_QT_adc0_coarse_freq: 0
      mask TypeOptions t226_QT_adc0_nyquist_zone: Zone 1 | Zone 2
      mask TypeOptions t226_QT_adc0_cal_mode: Mode 1 | Mode 2
      mask Callback t226_QT_adc1_enable: enable_adc_opt(gcb,226,1);
      mask TypeOptions t226_QT_adc1_digital_output: Real | I/Q
      mask Callback t226_QT_adc1_digital_output:
      | validate_digital_data(gcb,226,1,'QT');
      | update_axis_clk(gcb,226);
      mask TypeOptions t226_QT_adc1_dec_mode: 1x | 2x | 4x | 8x
      mask Callback t226_QT_adc1_dec_mode: update_axis_clk(gcb,226);
      mask TypeOptions t226_QT_adc1_sample_per_cycle: 1 | 2 | 3 | 4 | 5 | 6 | 7 | 8 | 9 | 10 | 11 | 12
      mask Callback t226_QT_adc1_sample_per_cycle: update_axis_clk_label(gcb,226);
      mask TypeOptions t226_QT_adc1_mixer_type: Bypassed
      mask Callback t226_QT_adc1_mixer_type: mixertype_callback(gcb,226,1,'QT');
      mask TypeOptions t226_QT_adc1_mixer_mode: Real -> Real
      mask Callback t226_QT_adc1_mixer_mode: mixer_callback(gcb,226,1,'QT')
      mask TypeOptions t226_QT_adc1_coarse_freq: 0
      mask TypeOptions t226_QT_adc1_nyquist_zone: Zone 1 | Zone 2
      mask TypeOptions t226_QT_adc1_cal_mode: Mode 1 | Mode 2
      mask Callback t226_QT_adc2_enable: enable_adc_opt(gcb,226,2);
      mask TypeOptions t226_QT_adc2_digital_output: Real | I/Q
      mask Callback t226_QT_adc2_digital_output:
      | validate_digital_data(gcb,226,2,'QT');
      | update_axis_clk(gcb,226);
      mask TypeOptions t226_QT_adc2_dec_mode: 1x | 2x | 4x | 8x
      mask Callback t226_QT_adc2_dec_mode: update_axis_clk(gcb,226);
      mask TypeOptions t226_QT_adc2_sample_per_cycle: 1 | 2 | 3 | 4 | 5 | 6 | 7 | 8 | 9 | 10 | 11 | 12
      mask Callback t226_QT_adc2_sample_per_cycle: update_axis_clk_label(gcb,226);
      mask TypeOptions t226_QT_adc2_mixer_type: Bypassed
      mask Callback t226_QT_adc2_mixer_type: mixertype_callback(gcb,226,2,'QT');
      mask TypeOptions t226_QT_adc2_mixer_mode: Real -> Real
      mask Callback t226_QT_adc2_mixer_mode: mixer_callback(gcb,226,2,'QT')
      mask TypeOptions t226_QT_adc2_coarse_freq: 0
      mask TypeOptions t226_QT_adc2_nyquist_zone: Zone 1 | Zone 2
      mask TypeOptions t226_QT_adc2_cal_mode: Mode 1 | Mode 2
      mask Callback t226_QT_adc3_enable: enable_adc_opt(gcb,226,3);
      mask TypeOptions t226_QT_adc3_digital_output: Real | I/Q
      mask Callback t226_QT_adc3_digital_output:
      | validate_digital_data(gcb,226,3,'QT');
      | update_axis_clk(gcb,226);
      mask TypeOptions t226_QT_adc3_dec_mode: 1x | 2x | 4x | 8x
      mask Callback t226_QT_adc3_dec_mode: update_axis_clk(gcb,226);
      mask TypeOptions t226_QT_adc3_sample_per_cycle: 1 | 2 | 3 | 4 | 5 | 6 | 7 | 8 | 9 | 10 | 11 | 12
      mask Callback t226_QT_adc3_sample_per_cycle: update_axis_clk_label(gcb,226);
      mask TypeOptions t226_QT_adc3_mixer_type: Bypassed
      mask Callback t226_QT_adc3_mixer_type: mixertype_callback(gcb,226,3,'QT');
      mask TypeOptions t226_QT_adc3_mixer_mode: Real -> Real
      mask Callback t226_QT_adc3_mixer_mode: mixer_callback(gcb,226,3,'QT')
      mask TypeOptions t226_QT_adc3_coarse_freq: 0
      mask TypeOptions t226_QT_adc3_nyquist_zone: Zone 1 | Zone 2
      mask TypeOptions t226_QT_adc3_cal_mode: Mode 1 | Mode 2
      mask Callback t226_DT_adc0_enable: enable_adc_opt(gcb,226,0);
      mask TypeOptions t226_DT_adc0_digital_output: Real | I/Q
      mask Callback t226_DT_adc0_digital_output:
      | validate_digital_data(gcb,226,0,'DT');
      | update_axis_clk(gcb,226);
      mask TypeOptions t226_DT_adc0_dec_mode: 1x | 2x | 4x | 8x
      mask Callback t226_DT_adc0_dec_mode: update_axis_clk(gcb,226);
      mask TypeOptions t226_DT_adc0_sample_per_cycle: 2 | 3 | 4 | 5 | 6 | 7 | 8
      mask Callback t226_DT_adc0_sample_per_cycle:
      | %update_axis_clk(gcb);
      | update_axis_clk_label(gcb,226);
      mask TypeOptions t226_DT_adc0_mixer_type: Bypassed
      mask Callback t226_DT_adc0_mixer_type: mixertype_callback(gcb,226,0,'DT');
      mask TypeOptions t226_DT_adc0_mixer_mode: Real -> Real
      mask Callback t226_DT_adc0_mixer_mode: mixer_callback(gcb,226,0,'DT');
      mask TypeOptions t226_DT_adc0_coarse_freq: 0
      mask TypeOptions t226_DT_adc0_nyquist_zone: Zone 1 | Zone 2
      mask TypeOptions t226_DT_adc0_cal_mode: Mode 1 | Mode 2
      mask Callback t226_DT_adc1_enable: enable_adc_opt(gcb,226,1);
      mask TypeOptions t226_DT_adc1_digital_output: Real | I/Q
      mask Callback t226_DT_adc1_digital_output:
      | validate_digital_data(gcb,226,1,'DT');
      | update_axis_clk(gcb,226);
      mask TypeOptions t226_DT_adc1_dec_mode: 1x | 2x | 4x | 8x
      mask Callback t226_DT_adc1_dec_mode: update_axis_clk(gcb,226);
      mask TypeOptions t226_DT_adc1_sample_per_cycle: 2 | 3 | 4 | 5 | 6 | 7 | 8
      mask Callback t226_DT_adc1_sample_per_cycle:
      | %update_axis_clk(gcb);
      | update_axis_clk_label(gcb,226);
      mask TypeOptions t226_DT_adc1_mixer_type: Bypassed
      mask Callback t226_DT_adc1_mixer_type: mixertype_callback(gcb,226,1,'DT');
      mask TypeOptions t226_DT_adc1_mixer_mode: Real -> Real
      mask Callback t226_DT_adc1_mixer_mode: mixer_callback(gcb,226,1,'DT');
      mask TypeOptions t226_DT_adc1_coarse_freq: 0
      mask TypeOptions t226_DT_adc1_nyquist_zone: Zone 1 | Zone 2
      mask TypeOptions t226_DT_adc1_cal_mode: Mode 1 | Mode 2
      mask Callback t227_sample_rate: update_rfdc_clocking(gcb,227);
      mask TypeOptions t227_clk_out: 125 | 62.5 | 31.25 | 15.625
      mask Callback t227_enable_pll:
      | %update_rfdc_clocking(gcb);
      | update_pll(gcb,227);
      mask TypeOptions t227_ref_clk: 923.077 | 857.143 | 800 | 750 | 705.882 | 666.667 | 631.579 | 600 | 571.429 | 545.455 | 521.739 | 500 | 480 | 461.538 | 444.444 | 428.571 | 413.793 | 400 | 387.097 | 375 | 363.636 | 352.941 | 342.857 | 333.333 | 324.324 | 315.789 | 307.692 | 300 | 292.683 | 285.714 | 279.07 | 272.727 | 266.667 | 260.87 | 255.319 | 250 | 244.898 | 240 | 235.294 | 230.769 | 226.415 | 222.222 | 218.182 | 214.286 | 210.526 | 206.897 | 203.39 | 200 | 196.721 | 193.548 | 190.476 | 187.5 | 184.615 | 181.818 | 179.104 | 176.471 | 173.913 | 171.429 | 169.014 | 166.667 | 164.384 | 162.162 | 160 | 157.895 | 155.844 | 153.846 | 151.899 | 150 | 148.148 | 146.341 | 144.578 | 142.857 | 141.176 | 139.535 | 137.931 | 136.364 | 134.831 | 133.333 | 131.868 | 130.435 | 129.032 | 127.66 | 126.316 | 125 | 123.711 | 122.449 | 121.212 | 120 | 118.812 | 117.647 | 116.505 | 115.385 | 114.286 | 113.208 | 112.15 | 111.111 | 110.092 | 109.091 | 108.108 | 107.143 | 106.195 | 105.263 | 104.348 | 103.448 | 102.564
      mask Callback t227_QT_adc0_enable: enable_adc_opt(gcb,227,0);
      mask TypeOptions t227_QT_adc0_digital_output: Real | I/Q
      mask Callback t227_QT_adc0_digital_output:
      | validate_digital_data(gcb,227,0,'QT');
      | update_axis_clk(gcb,227);
      mask TypeOptions t227_QT_adc0_dec_mode: 1x | 2x | 4x | 8x
      mask Callback t227_QT_adc0_dec_mode: update_axis_clk(gcb,227);
      mask TypeOptions t227_QT_adc0_sample_per_cycle: 1 | 2 | 3 | 4 | 5 | 6 | 7 | 8 | 9 | 10 | 11 | 12
      mask Callback t227_QT_adc0_sample_per_cycle:
      | %update_axis_clk(gcb);
      | update_axis_clk_label(gcb,227);
      mask TypeOptions t227_QT_adc0_mixer_type: Bypassed
      mask Callback t227_QT_adc0_mixer_type: mixertype_callback(gcb,227,0,'QT');
      mask TypeOptions t227_QT_adc0_mixer_mode: Real -> Real
      mask Callback t227_QT_adc0_mixer_mode: mixer_callback(gcb,227,0,'QT');
      mask TypeOptions t227_QT_adc0_coarse_freq: 0
      mask TypeOptions t227_QT_adc0_nyquist_zone: Zone 1 | Zone 2
      mask TypeOptions t227_QT_adc0_cal_mode: Mode 1 | Mode 2
      mask Callback t227_QT_adc1_enable: enable_adc_opt(gcb,227,1);
      mask TypeOptions t227_QT_adc1_digital_output: Real | I/Q
      mask Callback t227_QT_adc1_digital_output:
      | validate_digital_data(gcb,227,1,'QT');
      | update_axis_clk(gcb,227);
      mask TypeOptions t227_QT_adc1_dec_mode: 1x | 2x | 4x | 8x
      mask Callback t227_QT_adc1_dec_mode: update_axis_clk(gcb,227);
      mask TypeOptions t227_QT_adc1_sample_per_cycle: 1 | 2 | 3 | 4 | 5 | 6 | 7 | 8 | 9 | 10 | 11 | 12
      mask Callback t227_QT_adc1_sample_per_cycle: update_axis_clk_label(gcb,227);
      mask TypeOptions t227_QT_adc1_mixer_type: Bypassed
      mask Callback t227_QT_adc1_mixer_type: mixertype_callback(gcb,227,1,'QT');
      mask TypeOptions t227_QT_adc1_mixer_mode: Real -> Real
      mask Callback t227_QT_adc1_mixer_mode: mixer_callback(gcb,227,1,'QT')
      mask TypeOptions t227_QT_adc1_coarse_freq: 0
      mask TypeOptions t227_QT_adc1_nyquist_zone: Zone 1 | Zone 2
      mask TypeOptions t227_QT_adc1_cal_mode: Mode 1 | Mode 2
      mask Callback t227_QT_adc2_enable: enable_adc_opt(gcb,227,2);
      mask TypeOptions t227_QT_adc2_digital_output: Real | I/Q
      mask Callback t227_QT_adc2_digital_output:
      | validate_digital_data(gcb,227,2,'QT');
      | update_axis_clk(gcb,227);
      mask TypeOptions t227_QT_adc2_dec_mode: 1x | 2x | 4x | 8x
      mask Callback t227_QT_adc2_dec_mode: update_axis_clk(gcb,227);
      mask TypeOptions t227_QT_adc2_sample_per_cycle: 1 | 2 | 3 | 4 | 5 | 6 | 7 | 8 | 9 | 10 | 11 | 12
      mask Callback t227_QT_adc2_sample_per_cycle: update_axis_clk_label(gcb,227);
      mask TypeOptions t227_QT_adc2_mixer_type: Bypassed
      mask Callback t227_QT_adc2_mixer_type: mixertype_callback(gcb,227,2,'QT');
      mask TypeOptions t227_QT_adc2_mixer_mode: Real -> Real
      mask Callback t227_QT_adc2_mixer_mode: mixer_callback(gcb,227,2,'QT')
      mask TypeOptions t227_QT_adc2_coarse_freq: 0
      mask TypeOptions t227_QT_adc2_nyquist_zone: Zone 1 | Zone 2
      mask TypeOptions t227_QT_adc2_cal_mode: Mode 1 | Mode 2
      mask Callback t227_QT_adc3_enable: enable_adc_opt(gcb,227,3);
      mask TypeOptions t227_QT_adc3_digital_output: Real | I/Q
      mask Callback t227_QT_adc3_digital_output:
      | validate_digital_data(gcb,227,3,'QT');
      | update_axis_clk(gcb,227);
      mask TypeOptions t227_QT_adc3_dec_mode: 1x | 2x | 4x | 8x
      mask Callback t227_QT_adc3_dec_mode: update_axis_clk(gcb,227);
      mask TypeOptions t227_QT_adc3_sample_per_cycle: 1 | 2 | 3 | 4 | 5 | 6 | 7 | 8 | 9 | 10 | 11 | 12
      mask Callback t227_QT_adc3_sample_per_cycle: update_axis_clk_label(gcb,227);
      mask TypeOptions t227_QT_adc3_mixer_type: Bypassed
      mask Callback t227_QT_adc3_mixer_type: mixertype_callback(gcb,227,3,'QT');
      mask TypeOptions t227_QT_adc3_mixer_mode: Real -> Real
      mask Callback t227_QT_adc3_mixer_mode: mixer_callback(gcb,227,3,'QT')
      mask TypeOptions t227_QT_adc3_coarse_freq: 0
      mask TypeOptions t227_QT_adc3_nyquist_zone: Zone 1 | Zone 2
      mask TypeOptions t227_QT_adc3_cal_mode: Mode 1 | Mode 2
      mask Callback t227_DT_adc0_enable: enable_adc_opt(gcb,227,0);
      mask TypeOptions t227_DT_adc0_digital_output: Real | I/Q
      mask Callback t227_DT_adc0_digital_output:
      | validate_digital_data(gcb,227,0,'DT');
      | update_axis_clk(gcb,227);
      mask TypeOptions t227_DT_adc0_dec_mode: 1x | 2x | 4x | 8x
      mask Callback t227_DT_adc0_dec_mode: update_axis_clk(gcb,227);
      mask TypeOptions t227_DT_adc0_sample_per_cycle: 2 | 3 | 4 | 5 | 6 | 7 | 8
      mask Callback t227_DT_adc0_sample_per_cycle:
      | %update_axis_clk(gcb);
      | update_axis_clk_label(gcb,227);
      mask TypeOptions t227_DT_adc0_mixer_type: Bypassed
      mask Callback t227_DT_adc0_mixer_type: mixertype_callback(gcb,227,0,'DT');
      mask TypeOptions t227_DT_adc0_mixer_mode: Real -> Real
      mask Callback t227_DT_adc0_mixer_mode: mixer_callback(gcb,227,0,'DT');
      mask TypeOptions t227_DT_adc0_coarse_freq: 0
      mask TypeOptions t227_DT_adc0_nyquist_zone: Zone 1 | Zone 2
      mask TypeOptions t227_DT_adc0_cal_mode: Mode 1 | Mode 2
      mask Callback t227_DT_adc1_enable: enable_adc_opt(gcb,227,1);
      mask TypeOptions t227_DT_adc1_digital_output: Real | I/Q
      mask Callback t227_DT_adc1_digital_output:
      | validate_digital_data(gcb,227,1,'DT');
      | update_axis_clk(gcb,227);
      mask TypeOptions t227_DT_adc1_dec_mode: 1x | 2x | 4x | 8x
      mask Callback t227_DT_adc1_dec_mode: update_axis_clk(gcb,227);
      mask TypeOptions t227_DT_adc1_sample_per_cycle: 2 | 3 | 4 | 5 | 6 | 7 | 8
      mask Callback t227_DT_adc1_sample_per_cycle:
      | %update_axis_clk(gcb);
      | update_axis_clk_label(gcb,227);
      mask TypeOptions t227_DT_adc1_mixer_type: Bypassed
      mask Callback t227_DT_adc1_mixer_type: mixertype_callback(gcb,227,1,'DT');
      mask TypeOptions t227_DT_adc1_mixer_mode: Real -> Real
      mask Callback t227_DT_adc1_mixer_mode: mixer_callback(gcb,227,1,'DT');
      mask TypeOptions t227_DT_adc1_coarse_freq: 0
      mask TypeOptions t227_DT_adc1_nyquist_zone: Zone 1 | Zone 2
      mask TypeOptions t227_DT_adc1_cal_mode: Mode 1 | Mode 2
      mask Callback t228_sample_rate: update_rfdc_clocking(gcb,228);
      mask TypeOptions t228_clk_out: 125 | 62.5 | 31.25 | 15.625
      mask Callback t228_enable_pll:
      | %update_rfdc_clocking(gcb);
      | update_pll(gcb,228);
      mask TypeOptions t228_ref_clk: 923.077 | 857.143 | 800 | 750 | 705.882 | 666.667 | 631.579 | 600 | 571.429 | 545.455 | 521.739 | 500 | 480 | 461.538 | 444.444 | 428.571 | 413.793 | 400 | 387.097 | 375 | 363.636 | 352.941 | 342.857 | 333.333 | 324.324 | 315.789 | 307.692 | 300 | 292.683 | 285.714 | 279.07 | 272.727 | 266.667 | 260.87 | 255.319 | 250 | 244.898 | 240 | 235.294 | 230.769 | 226.415 | 222.222 | 218.182 | 214.286 | 210.526 | 206.897 | 203.39 | 200 | 196.721 | 193.548 | 190.476 | 187.5 | 184.615 | 181.818 | 179.104 | 176.471 | 173.913 | 171.429 | 169.014 | 166.667 | 164.384 | 162.162 | 160 | 157.895 | 155.844 | 153.846 | 151.899 | 150 | 148.148 | 146.341 | 144.578 | 142.857 | 141.176 | 139.535 | 137.931 | 136.364 | 134.831 | 133.333 | 131.868 | 130.435 | 129.032 | 127.66 | 126.316 | 125 | 123.711 | 122.449 | 121.212 | 120 | 118.812 | 117.647 | 116.505 | 115.385 | 114.286 | 113.208 | 112.15 | 111.111 | 110.092 | 109.091 | 108.108 | 107.143 | 106.195 | 105.263 | 104.348 | 103.448 | 102.564
      mask Callback t228_QT_dac0_enable: enable_dac_opt(gcb,228,0);
      mask TypeOptions t228_QT_dac0_analog_output: Real | I/Q
      mask Callback t228_QT_dac0_analog_output:
      | validate_analog_data(gcb,228,0,'QT');
      | update_axis_clk(gcb,228);
      mask TypeOptions t228_QT_dac0_inter_mode: 1x | 2x | 4x | 8x | 10x | 12x | 16x | 20x | 24x | 40x
      mask Callback t228_QT_dac0_inter_mode: update_axis_clk(gcb,228);
      mask TypeOptions t228_QT_dac0_sample_per_cycle: 1 | 2 | 3 | 4 | 5 | 6 | 7 | 8 | 9 | 10 | 11 | 12 | 13 | 14 | 15 | 16
      mask Callback t228_QT_dac0_sample_per_cycle:
      | %update_axis_clk(gcb);
      | update_axis_clk_label(gcb,228);
      mask TypeOptions t228_QT_dac0_datapath_mode: DUC 0 to Fs/2 | DUC 0 to Fs/4 | DUC Fs/4 to Fs/2 | No DUC 0 to Fs/2
      mask TypeOptions t228_QT_dac0_mixer_type: Bypassed
      mask Callback t228_QT_dac0_mixer_type: mixertype_callback(gcb,228,0,'QT');
      mask TypeOptions t228_QT_dac0_mixer_mode: Real -> Real | I/Q -> Real
      mask Callback t228_QT_dac0_mixer_mode: mixer_callback(gcb,228,0,'QT');
      mask TypeOptions t228_QT_dac0_coarse_freq: 0
      mask TypeOptions t228_QT_dac0_nyquist_zone: Zone 1 | Zone 2
      mask TypeOptions t228_QT_dac0_decode_mode: SNR Optimized | Linearity Optimized
      mask Callback t228_QT_dac1_enable: enable_dac_opt(gcb,228,1);
      mask TypeOptions t228_QT_dac1_analog_output: Real | I/Q
      mask Callback t228_QT_dac1_analog_output:
      | validate_analog_data(gcb,228,1,'QT');
      | update_axis_clk(gcb,228);
      mask TypeOptions t228_QT_dac1_inter_mode: 1x | 2x | 4x | 8x | 10x | 12x | 16x | 20x | 24x | 40x
      mask Callback t228_QT_dac1_inter_mode: update_axis_clk(gcb,228);
      mask TypeOptions t228_QT_dac1_sample_per_cycle: 1 | 2 | 3 | 4 | 5 | 6 | 7 | 8 | 9 | 10 | 11 | 12 | 13 | 14 | 15 | 16
      mask Callback t228_QT_dac1_sample_per_cycle: update_axis_clk_label(gcb,228);
      mask TypeOptions t228_QT_dac1_datapath_mode: DUC 0 to Fs/2 | DUC 0 to Fs/4 | DUC Fs/4 to Fs/2 | No DUC 0 to Fs/2
      mask TypeOptions t228_QT_dac1_mixer_type: Bypassed
      mask Callback t228_QT_dac1_mixer_type: mixertype_callback(gcb,228,1,'QT');
      mask TypeOptions t228_QT_dac1_mixer_mode: Real -> Real | I/Q -> Real
      mask Callback t228_QT_dac1_mixer_mode: mixer_callback(gcb,228,1,'QT')
      mask TypeOptions t228_QT_dac1_coarse_freq: 0
      mask TypeOptions t228_QT_dac1_nyquist_zone: Zone 1 | Zone 2
      mask TypeOptions t228_QT_dac1_decode_mode: SNR Optimized | Linearity Optimized
      mask Callback t228_QT_dac2_enable: enable_dac_opt(gcb,228,2);
      mask TypeOptions t228_QT_dac2_analog_output: Real | I/Q
      mask Callback t228_QT_dac2_analog_output:
      | validate_analog_data(gcb,228,2,'QT');
      | update_axis_clk(gcb,228);
      mask TypeOptions t228_QT_dac2_inter_mode: 1x | 2x | 4x | 8x | 10x | 12x | 16x | 20x | 24x | 40x
      mask Callback t228_QT_dac2_inter_mode: update_axis_clk(gcb,228);
      mask TypeOptions t228_QT_dac2_sample_per_cycle: 1 | 2 | 3 | 4 | 5 | 6 | 7 | 8 | 9 | 10 | 11 | 12 | 13 | 14 | 15 | 16
      mask Callback t228_QT_dac2_sample_per_cycle: update_axis_clk_label(gcb,228);
      mask TypeOptions t228_QT_dac2_datapath_mode: DUC 0 to Fs/2 | DUC 0 to Fs/4 | DUC Fs/4 to Fs/2 | No DUC 0 to Fs/2
      mask TypeOptions t228_QT_dac2_mixer_type: Bypassed
      mask Callback t228_QT_dac2_mixer_type: mixertype_callback(gcb,228,2,'QT');
      mask TypeOptions t228_QT_dac2_mixer_mode: Real -> Real | I/Q -> Real
      mask Callback t228_QT_dac2_mixer_mode: mixer_callback(gcb,228,2,'QT')
      mask TypeOptions t228_QT_dac2_coarse_freq: 0
      mask TypeOptions t228_QT_dac2_nyquist_zone: Zone 1 | Zone 2
      mask TypeOptions t228_QT_dac2_decode_mode: SNR Optimized | Linearity Optimized
      mask Callback t228_QT_dac3_enable: enable_dac_opt(gcb,228,3);
      mask TypeOptions t228_QT_dac3_analog_output: Real | I/Q
      mask Callback t228_QT_dac3_analog_output:
      | validate_analog_data(gcb,228,3,'QT');
      | update_axis_clk(gcb,228);
      mask TypeOptions t228_QT_dac3_inter_mode: 1x | 2x | 4x | 8x | 10x | 12x | 16x | 20x | 24x | 40x
      mask Callback t228_QT_dac3_inter_mode: update_axis_clk(gcb,228);
      mask TypeOptions t228_QT_dac3_sample_per_cycle: 1 | 2 | 3 | 4 | 5 | 6 | 7 | 8 | 9 | 10 | 11 | 12 | 13 | 14 | 15 | 16
      mask Callback t228_QT_dac3_sample_per_cycle: update_axis_clk_label(gcb,228);
      mask TypeOptions t228_QT_dac3_datapath_mode: DUC 0 to Fs/2 | DUC 0 to Fs/4 | DUC Fs/4 to Fs/2 | No DUC 0 to Fs/2
      mask TypeOptions t228_QT_dac3_mixer_type: Bypassed
      mask Callback t228_QT_dac3_mixer_type: mixertype_callback(gcb,228,3,'QT');
      mask TypeOptions t228_QT_dac3_mixer_mode: Real -> Real | I/Q -> Real
      mask Callback t228_QT_dac3_mixer_mode: mixer_callback(gcb,228,3,'QT')
      mask TypeOptions t228_QT_dac3_coarse_freq: 0
      mask TypeOptions t228_QT_dac3_nyquist_zone: Zone 1 | Zone 2
      mask TypeOptions t228_QT_dac3_decode_mode: SNR Optimized | Linearity Optimized
      mask Callback t228_DT_dac0_enable: enable_dac_opt(gcb,228,0);
      mask TypeOptions t228_DT_dac0_analog_output: Real | I/Q
      mask Callback t228_DT_dac0_analog_output:
      | validate_analog_data(gcb,228,0,'DT');
      | update_axis_clk(gcb,228);
      mask TypeOptions t228_DT_dac0_inter_mode: 1x | 2x | 4x | 8x
      mask Callback t228_DT_dac0_inter_mode: update_axis_clk(gcb,228);
      mask TypeOptions t228_DT_dac0_sample_per_cycle: 2 | 3 | 4 | 5 | 6 | 7 | 8
      mask Callback t228_DT_dac0_sample_per_cycle:
      | %update_axis_clk(gcb);
      | update_axis_clk_label(gcb,228);
      mask TypeOptions t228_DT_dac0_mixer_type: Fine | Coarse
      mask Callback t228_DT_dac0_mixer_type: mixertype_callback(gcb,228,0,'DT');
      mask TypeOptions t228_DT_dac0_mixer_mode: I/Q -> I/Q
      mask Callback t228_DT_dac0_mixer_mode: mixer_callback(gcb,228,0,'DT');
      mask TypeOptions t228_DT_dac0_coarse_freq: 0
      mask TypeOptions t228_DT_dac0_nyquist_zone: Zone 1 | Zone 2
      mask TypeOptions t228_DT_dac0_decode_mode: SNR Optimized | Linearity Optimized
      mask Callback t228_DT_dac1_enable: enable_dac_opt(gcb,228,1);
      mask TypeOptions t228_DT_dac1_analog_output: Real | I/Q
      mask Callback t228_DT_dac1_analog_output:
      | validate_analog_data(gcb,228,1,'DT');
      | update_axis_clk(gcb,228);
      mask TypeOptions t228_DT_dac1_inter_mode: 1x | 2x | 4x | 8x
      mask Callback t228_DT_dac1_inter_mode: update_axis_clk(gcb,228);
      mask TypeOptions t228_DT_dac1_sample_per_cycle: 2 | 3 | 4 | 5 | 6 | 7 | 8
      mask Callback t228_DT_dac1_sample_per_cycle:
      | %update_axis_clk(gcb);
      | update_axis_clk_label(gcb,228);
      mask TypeOptions t228_DT_dac1_mixer_type: Off
      mask Callback t228_DT_dac1_mixer_type: mixertype_callback(gcb,228,1,'DT');
      mask TypeOptions t228_DT_dac1_mixer_mode: Off
      mask Callback t228_DT_dac1_mixer_mode: mixer_callback(gcb,228,1,'DT');
      mask TypeOptions t228_DT_dac1_coarse_freq: 0
      mask TypeOptions t228_DT_dac1_nyquist_zone: Zone 1 | Zone 2
      mask TypeOptions t228_DT_dac1_decode_mode: SNR Optimized | Linearity Optimized
      mask Callback t228_DT_dac2_enable: enable_dac_opt(gcb,228,2);
      mask TypeOptions t228_DT_dac2_analog_output: Real | I/Q
      mask Callback t228_DT_dac2_analog_output:
      | validate_analog_data(gcb,228,2,'DT');
      | update_axis_clk(gcb,228);
      mask TypeOptions t228_DT_dac2_inter_mode: 1x | 2x | 4x | 8x
      mask Callback t228_DT_dac2_inter_mode: update_axis_clk(gcb,228);
      mask TypeOptions t228_DT_dac2_sample_per_cycle: 2 | 3 | 4 | 5 | 6 | 7 | 8
      mask Callback t228_DT_dac2_sample_per_cycle:
      | %update_axis_clk(gcb);
      | update_axis_clk_label(gcb,228);
      mask TypeOptions t228_DT_dac2_mixer_type: Bypassed
      mask Callback t228_DT_dac2_mixer_type: mixertype_callback(gcb,228,2,'DT');
      mask TypeOptions t228_DT_dac2_mixer_mode: Real -> Real | I/Q -> Real
      mask Callback t228_DT_dac2_mixer_mode: mixer_callback(gcb,228,2,'DT');
      mask TypeOptions t228_DT_dac2_coarse_freq: 0
      mask TypeOptions t228_DT_dac2_nyquist_zone: Zone 1 | Zone 2
      mask TypeOptions t228_DT_dac2_decode_mode: SNR Optimized | Linearity Optimized
      mask Callback t228_DT_dac3_enable: enable_dac_opt(gcb,228,3);
      mask TypeOptions t228_DT_dac3_analog_output: Real | I/Q
      mask Callback t228_DT_dac3_analog_output:
      | validate_analog_data(gcb,228,3,'DT');
      | update_axis_clk(gcb,228);
      mask TypeOptions t228_DT_dac3_inter_mode: 1x | 2x | 4x | 8x
      mask Callback t228_DT_dac3_inter_mode: update_axis_clk(gcb,228);
      mask TypeOptions t228_DT_dac3_sample_per_cycle: 2 | 3 | 4 | 5 | 6 | 7 | 8
      mask Callback t228_DT_dac3_sample_per_cycle:
      | %update_axis_clk(gcb);
      | update_axis_clk_label(gcb,228);
      mask TypeOptions t228_DT_dac3_mixer_type: Bypassed
      mask Callback t228_DT_dac3_mixer_type: mixertype_callback(gcb,228,3,'DT');
      mask TypeOptions t228_DT_dac3_mixer_mode: Real -> Real | I/Q -> Real
      mask Callback t228_DT_dac3_mixer_mode: mixer_callback(gcb,228,3,'DT');
      mask TypeOptions t228_DT_dac3_coarse_freq: 0
      mask TypeOptions t228_DT_dac3_nyquist_zone: Zone 1 | Zone 2
      mask TypeOptions t228_DT_dac3_decode_mode: SNR Optimized | Linearity Optimized
      mask Callback t229_sample_rate: update_rfdc_clocking(gcb,229);
      mask TypeOptions t229_clk_out: 125 | 62.5 | 31.25 | 15.625
      mask Callback t229_enable_pll:
      | %update_rfdc_clocking(gcb);
      | update_pll(gcb,229);
      mask TypeOptions t229_ref_clk: 923.077 | 857.143 | 800 | 750 | 705.882 | 666.667 | 631.579 | 600 | 571.429 | 545.455 | 521.739 | 500 | 480 | 461.538 | 444.444 | 428.571 | 413.793 | 400 | 387.097 | 375 | 363.636 | 352.941 | 342.857 | 333.333 | 324.324 | 315.789 | 307.692 | 300 | 292.683 | 285.714 | 279.07 | 272.727 | 266.667 | 260.87 | 255.319 | 250 | 244.898 | 240 | 235.294 | 230.769 | 226.415 | 222.222 | 218.182 | 214.286 | 210.526 | 206.897 | 203.39 | 200 | 196.721 | 193.548 | 190.476 | 187.5 | 184.615 | 181.818 | 179.104 | 176.471 | 173.913 | 171.429 | 169.014 | 166.667 | 164.384 | 162.162 | 160 | 157.895 | 155.844 | 153.846 | 151.899 | 150 | 148.148 | 146.341 | 144.578 | 142.857 | 141.176 | 139.535 | 137.931 | 136.364 | 134.831 | 133.333 | 131.868 | 130.435 | 129.032 | 127.66 | 126.316 | 125 | 123.711 | 122.449 | 121.212 | 120 | 118.812 | 117.647 | 116.505 | 115.385 | 114.286 | 113.208 | 112.15 | 111.111 | 110.092 | 109.091 | 108.108 | 107.143 | 106.195 | 105.263 | 104.348 | 103.448 | 102.564
      mask Callback t229_QT_dac0_enable: enable_dac_opt(gcb,229,0);
      mask TypeOptions t229_QT_dac0_analog_output: Real | I/Q
      mask Callback t229_QT_dac0_analog_output:
      | validate_analog_data(gcb,229,0,'QT');
      | update_axis_clk(gcb,229);
      mask TypeOptions t229_QT_dac0_inter_mode: 1x | 2x | 4x | 8x | 10x | 12x | 16x | 20x | 24x | 40x
      mask Callback t229_QT_dac0_inter_mode: update_axis_clk(gcb,229);
      mask TypeOptions t229_QT_dac0_sample_per_cycle: 1 | 2 | 3 | 4 | 5 | 6 | 7 | 8 | 9 | 10 | 11 | 12 | 13 | 14 | 15 | 16
      mask Callback t229_QT_dac0_sample_per_cycle:
      | %update_axis_clk(gcb);
      | update_axis_clk_label(gcb,229);
      mask TypeOptions t229_QT_dac0_datapath_mode: DUC 0 to Fs/2 | DUC 0 to Fs/4 | DUC Fs/4 to Fs/2 | No DUC 0 to Fs/2
      mask TypeOptions t229_QT_dac0_mixer_type: Bypassed
      mask Callback t229_QT_dac0_mixer_type: mixertype_callback(gcb,229,0,'QT');
      mask TypeOptions t229_QT_dac0_mixer_mode: Real -> Real | I/Q -> Real
      mask Callback t229_QT_dac0_mixer_mode: mixer_callback(gcb,229,0,'QT');
      mask TypeOptions t229_QT_dac0_coarse_freq: 0
      mask TypeOptions t229_QT_dac0_nyquist_zone: Zone 1 | Zone 2
      mask TypeOptions t229_QT_dac0_decode_mode: SNR Optimized | Linearity Optimized
      mask Callback t229_QT_dac1_enable: enable_dac_opt(gcb,229,1);
      mask TypeOptions t229_QT_dac1_analog_output: Real | I/Q
      mask Callback t229_QT_dac1_analog_output:
      | validate_analog_data(gcb,229,1,'QT');
      | update_axis_clk(gcb,229);
      mask TypeOptions t229_QT_dac1_inter_mode: 1x | 2x | 4x | 8x | 10x | 12x | 16x | 20x | 24x | 40x
      mask Callback t229_QT_dac1_inter_mode: update_axis_clk(gcb,229);
      mask TypeOptions t229_QT_dac1_sample_per_cycle: 1 | 2 | 3 | 4 | 5 | 6 | 7 | 8 | 9 | 10 | 11 | 12 | 13 | 14 | 15 | 16
      mask Callback t229_QT_dac1_sample_per_cycle: update_axis_clk_label(gcb,229);
      mask TypeOptions t229_QT_dac1_datapath_mode: DUC 0 to Fs/2 | DUC 0 to Fs/4 | DUC Fs/4 to Fs/2 | No DUC 0 to Fs/2
      mask TypeOptions t229_QT_dac1_mixer_type: Bypassed
      mask Callback t229_QT_dac1_mixer_type: mixertype_callback(gcb,229,1,'QT');
      mask TypeOptions t229_QT_dac1_mixer_mode: Real -> Real | I/Q -> Real
      mask Callback t229_QT_dac1_mixer_mode: mixer_callback(gcb,229,1,'QT')
      mask TypeOptions t229_QT_dac1_coarse_freq: 0
      mask TypeOptions t229_QT_dac1_nyquist_zone: Zone 1 | Zone 2
      mask TypeOptions t229_QT_dac1_decode_mode: SNR Optimized | Linearity Optimized
      mask Callback t229_QT_dac2_enable: enable_dac_opt(gcb,229,2);
      mask TypeOptions t229_QT_dac2_analog_output: Real | I/Q
      mask Callback t229_QT_dac2_analog_output:
      | validate_analog_data(gcb,229,2,'QT');
      | update_axis_clk(gcb,229);
      mask TypeOptions t229_QT_dac2_inter_mode: 1x | 2x | 4x | 8x | 10x | 12x | 16x | 20x | 24x | 40x
      mask Callback t229_QT_dac2_inter_mode: update_axis_clk(gcb,229);
      mask TypeOptions t229_QT_dac2_sample_per_cycle: 1 | 2 | 3 | 4 | 5 | 6 | 7 | 8 | 9 | 10 | 11 | 12 | 13 | 14 | 15 | 16
      mask Callback t229_QT_dac2_sample_per_cycle: update_axis_clk_label(gcb,229);
      mask TypeOptions t229_QT_dac2_datapath_mode: DUC 0 to Fs/2 | DUC 0 to Fs/4 | DUC Fs/4 to Fs/2 | No DUC 0 to Fs/2
      mask TypeOptions t229_QT_dac2_mixer_type: Bypassed
      mask Callback t229_QT_dac2_mixer_type: mixertype_callback(gcb,229,2,'QT');
      mask TypeOptions t229_QT_dac2_mixer_mode: Real -> Real | I/Q -> Real
      mask Callback t229_QT_dac2_mixer_mode: mixer_callback(gcb,229,2,'QT')
      mask TypeOptions t229_QT_dac2_coarse_freq: 0
      mask TypeOptions t229_QT_dac2_nyquist_zone: Zone 1 | Zone 2
      mask TypeOptions t229_QT_dac2_decode_mode: SNR Optimized | Linearity Optimized
      mask Callback t229_QT_dac3_enable: enable_dac_opt(gcb,229,3);
      mask TypeOptions t229_QT_dac3_analog_output: Real | I/Q
      mask Callback t229_QT_dac3_analog_output:
      | validate_analog_data(gcb,229,3,'QT');
      | update_axis_clk(gcb,229);
      mask TypeOptions t229_QT_dac3_inter_mode: 1x | 2x | 4x | 8x | 10x | 12x | 16x | 20x | 24x | 40x
      mask Callback t229_QT_dac3_inter_mode: update_axis_clk(gcb,229);
      mask TypeOptions t229_QT_dac3_sample_per_cycle: 1 | 2 | 3 | 4 | 5 | 6 | 7 | 8 | 9 | 10 | 11 | 12 | 13 | 14 | 15 | 16
      mask Callback t229_QT_dac3_sample_per_cycle: update_axis_clk_label(gcb,229);
      mask TypeOptions t229_QT_dac3_datapath_mode: DUC 0 to Fs/2 | DUC 0 to Fs/4 | DUC Fs/4 to Fs/2 | No DUC 0 to Fs/2
      mask TypeOptions t229_QT_dac3_mixer_type: Bypassed
      mask Callback t229_QT_dac3_mixer_type: mixertype_callback(gcb,229,3,'QT');
      mask TypeOptions t229_QT_dac3_mixer_mode: Real -> Real | I/Q -> Real
      mask Callback t229_QT_dac3_mixer_mode: mixer_callback(gcb,229,3,'QT')
      mask TypeOptions t229_QT_dac3_coarse_freq: 0
      mask TypeOptions t229_QT_dac3_nyquist_zone: Zone 1 | Zone 2
      mask TypeOptions t229_QT_dac3_decode_mode: SNR Optimized | Linearity Optimized
      mask Callback t229_DT_dac0_enable: enable_dac_opt(gcb,229,0);
      mask TypeOptions t229_DT_dac0_analog_output: Real | I/Q
      mask Callback t229_DT_dac0_analog_output:
      | validate_analog_data(gcb,229,0,'DT');
      | update_axis_clk(gcb,229);
      mask TypeOptions t229_DT_dac0_inter_mode: 1x | 2x | 4x | 8x
      mask Callback t229_DT_dac0_inter_mode: update_axis_clk(gcb,229);
      mask TypeOptions t229_DT_dac0_sample_per_cycle: 2 | 3 | 4 | 5 | 6 | 7 | 8
      mask Callback t229_DT_dac0_sample_per_cycle:
      | %update_axis_clk(gcb);
      | update_axis_clk_label(gcb,229);
      mask TypeOptions t229_DT_dac0_mixer_type: Bypassed
      mask Callback t229_DT_dac0_mixer_type: mixertype_callback(gcb,229,0,'DT');
      mask TypeOptions t229_DT_dac0_mixer_mode: Real -> Real | I/Q -> Real
      mask Callback t229_DT_dac0_mixer_mode: mixer_callback(gcb,229,0,'DT');
      mask TypeOptions t229_DT_dac0_coarse_freq: 0
      mask TypeOptions t229_DT_dac0_nyquist_zone: Zone 1 | Zone 2
      mask TypeOptions t229_DT_dac0_decode_mode: SNR Optimized | Linearity Optimized
      mask Callback t229_DT_dac1_enable: enable_dac_opt(gcb,229,1);
      mask TypeOptions t229_DT_dac1_analog_output: Real | I/Q
      mask Callback t229_DT_dac1_analog_output:
      | validate_analog_data(gcb,229,1,'DT');
      | update_axis_clk(gcb,229);
      mask TypeOptions t229_DT_dac1_inter_mode: 1x | 2x | 4x | 8x
      mask Callback t229_DT_dac1_inter_mode: update_axis_clk(gcb,229);
      mask TypeOptions t229_DT_dac1_sample_per_cycle: 2 | 3 | 4 | 5 | 6 | 7 | 8
      mask Callback t229_DT_dac1_sample_per_cycle:
      | %update_axis_clk(gcb);
      | update_axis_clk_label(gcb,229);
      mask TypeOptions t229_DT_dac1_mixer_type: Bypassed
      mask Callback t229_DT_dac1_mixer_type: mixertype_callback(gcb,229,1,'DT');
      mask TypeOptions t229_DT_dac1_mixer_mode: Real -> Real | I/Q -> Real
      mask Callback t229_DT_dac1_mixer_mode: mixer_callback(gcb,229,1,'DT');
      mask TypeOptions t229_DT_dac1_coarse_freq: 0
      mask TypeOptions t229_DT_dac1_nyquist_zone: Zone 1 | Zone 2
      mask TypeOptions t229_DT_dac1_decode_mode: SNR Optimized | Linearity Optimized
      mask Callback t229_DT_dac2_enable: enable_dac_opt(gcb,229,2);
      mask TypeOptions t229_DT_dac2_analog_output: Real | I/Q
      mask Callback t229_DT_dac2_analog_output:
      | validate_analog_data(gcb,229,2,'DT');
      | update_axis_clk(gcb,229);
      mask TypeOptions t229_DT_dac2_inter_mode: 1x | 2x | 4x | 8x
      mask Callback t229_DT_dac2_inter_mode: update_axis_clk(gcb,229);
      mask TypeOptions t229_DT_dac2_sample_per_cycle: 2 | 3 | 4 | 5 | 6 | 7 | 8
      mask Callback t229_DT_dac2_sample_per_cycle:
      | %update_axis_clk(gcb);
      | update_axis_clk_label(gcb,229);
      mask TypeOptions t229_DT_dac2_mixer_type: Bypassed
      mask Callback t229_DT_dac2_mixer_type: mixertype_callback(gcb,229,2,'DT');
      mask TypeOptions t229_DT_dac2_mixer_mode: Real -> Real | I/Q -> Real
      mask Callback t229_DT_dac2_mixer_mode: mixer_callback(gcb,229,2,'DT');
      mask TypeOptions t229_DT_dac2_coarse_freq: 0
      mask TypeOptions t229_DT_dac2_nyquist_zone: Zone 1 | Zone 2
      mask TypeOptions t229_DT_dac2_decode_mode: SNR Optimized | Linearity Optimized
      mask Callback t229_DT_dac3_enable: enable_dac_opt(gcb,229,3);
      mask TypeOptions t229_DT_dac3_analog_output: Real | I/Q
      mask Callback t229_DT_dac3_analog_output:
      | validate_analog_data(gcb,229,3,'DT');
      | update_axis_clk(gcb,229);
      mask TypeOptions t229_DT_dac3_inter_mode: 1x | 2x | 4x | 8x
      mask Callback t229_DT_dac3_inter_mode: update_axis_clk(gcb,229);
      mask TypeOptions t229_DT_dac3_sample_per_cycle: 2 | 3 | 4 | 5 | 6 | 7 | 8
      mask Callback t229_DT_dac3_sample_per_cycle:
      | %update_axis_clk(gcb);
      | update_axis_clk_label(gcb,229);
      mask TypeOptions t229_DT_dac3_mixer_type: Bypassed
      mask Callback t229_DT_dac3_mixer_type: mixertype_callback(gcb,229,3,'DT');
      mask TypeOptions t229_DT_dac3_mixer_mode: Real -> Real | I/Q -> Real
      mask Callback t229_DT_dac3_mixer_mode: mixer_callback(gcb,229,3,'DT');
      mask TypeOptions t229_DT_dac3_coarse_freq: 0
      mask TypeOptions t229_DT_dac3_nyquist_zone: Zone 1 | Zone 2
      mask TypeOptions t229_DT_dac3_decode_mode: SNR Optimized | Linearity Optimized
      mask Callback t230_sample_rate: update_rfdc_clocking(gcb,230);
      mask TypeOptions t230_clk_out: 125 | 62.5 | 31.25 | 15.625
      mask Callback t230_enable_pll:
      | %update_rfdc_clocking(gcb);
      | update_pll(gcb,230);
      mask TypeOptions t230_ref_clk: 923.077 | 857.143 | 800 | 750 | 705.882 | 666.667 | 631.579 | 600 | 571.429 | 545.455 | 521.739 | 500 | 480 | 461.538 | 444.444 | 428.571 | 413.793 | 400 | 387.097 | 375 | 363.636 | 352.941 | 342.857 | 333.333 | 324.324 | 315.789 | 307.692 | 300 | 292.683 | 285.714 | 279.07 | 272.727 | 266.667 | 260.87 | 255.319 | 250 | 244.898 | 240 | 235.294 | 230.769 | 226.415 | 222.222 | 218.182 | 214.286 | 210.526 | 206.897 | 203.39 | 200 | 196.721 | 193.548 | 190.476 | 187.5 | 184.615 | 181.818 | 179.104 | 176.471 | 173.913 | 171.429 | 169.014 | 166.667 | 164.384 | 162.162 | 160 | 157.895 | 155.844 | 153.846 | 151.899 | 150 | 148.148 | 146.341 | 144.578 | 142.857 | 141.176 | 139.535 | 137.931 | 136.364 | 134.831 | 133.333 | 131.868 | 130.435 | 129.032 | 127.66 | 126.316 | 125 | 123.711 | 122.449 | 121.212 | 120 | 118.812 | 117.647 | 116.505 | 115.385 | 114.286 | 113.208 | 112.15 | 111.111 | 110.092 | 109.091 | 108.108 | 107.143 | 106.195 | 105.263 | 104.348 | 103.448 | 102.564
      mask Callback t230_QT_dac0_enable: enable_dac_opt(gcb,230,0);
      mask TypeOptions t230_QT_dac0_analog_output: Real | I/Q
      mask Callback t230_QT_dac0_analog_output:
      | validate_analog_data(gcb,230,0,'QT');
      | update_axis_clk(gcb,230);
      mask TypeOptions t230_QT_dac0_inter_mode: 1x | 2x | 4x | 8x | 10x | 12x | 16x | 20x | 24x | 40x
      mask Callback t230_QT_dac0_inter_mode: update_axis_clk(gcb,230);
      mask TypeOptions t230_QT_dac0_sample_per_cycle: 1 | 2 | 3 | 4 | 5 | 6 | 7 | 8 | 9 | 10 | 11 | 12 | 13 | 14 | 15 | 16
      mask Callback t230_QT_dac0_sample_per_cycle:
      | %update_axis_clk(gcb);
      | update_axis_clk_label(gcb,230);
      mask TypeOptions t230_QT_dac0_datapath_mode: DUC 0 to Fs/2 | DUC 0 to Fs/4 | DUC Fs/4 to Fs/2 | No DUC 0 to Fs/2
      mask TypeOptions t230_QT_dac0_mixer_type: Bypassed
      mask Callback t230_QT_dac0_mixer_type: mixertype_callback(gcb,230,0,'QT');
      mask TypeOptions t230_QT_dac0_mixer_mode: Real -> Real | I/Q -> Real
      mask Callback t230_QT_dac0_mixer_mode: mixer_callback(gcb,230,0,'QT');
      mask TypeOptions t230_QT_dac0_coarse_freq: 0
      mask TypeOptions t230_QT_dac0_nyquist_zone: Zone 1 | Zone 2
      mask TypeOptions t230_QT_dac0_decode_mode: SNR Optimized | Linearity Optimized
      mask Callback t230_QT_dac1_enable: enable_dac_opt(gcb,230,1);
      mask TypeOptions t230_QT_dac1_analog_output: Real | I/Q
      mask Callback t230_QT_dac1_analog_output:
      | validate_analog_data(gcb,230,1,'QT');
      | update_axis_clk(gcb,230);
      mask TypeOptions t230_QT_dac1_inter_mode: 1x | 2x | 4x | 8x | 10x | 12x | 16x | 20x | 24x | 40x
      mask Callback t230_QT_dac1_inter_mode: update_axis_clk(gcb,230);
      mask TypeOptions t230_QT_dac1_sample_per_cycle: 1 | 2 | 3 | 4 | 5 | 6 | 7 | 8 | 9 | 10 | 11 | 12 | 13 | 14 | 15 | 16
      mask Callback t230_QT_dac1_sample_per_cycle: update_axis_clk_label(gcb,230);
      mask TypeOptions t230_QT_dac1_datapath_mode: DUC 0 to Fs/2 | DUC 0 to Fs/4 | DUC Fs/4 to Fs/2 | No DUC 0 to Fs/2
      mask TypeOptions t230_QT_dac1_mixer_type: Bypassed
      mask Callback t230_QT_dac1_mixer_type: mixertype_callback(gcb,230,1,'QT');
      mask TypeOptions t230_QT_dac1_mixer_mode: Real -> Real | I/Q -> Real
      mask Callback t230_QT_dac1_mixer_mode: mixer_callback(gcb,230,1,'QT')
      mask TypeOptions t230_QT_dac1_coarse_freq: 0
      mask TypeOptions t230_QT_dac1_nyquist_zone: Zone 1 | Zone 2
      mask TypeOptions t230_QT_dac1_decode_mode: SNR Optimized | Linearity Optimized
      mask Callback t230_QT_dac2_enable: enable_dac_opt(gcb,230,2);
      mask TypeOptions t230_QT_dac2_analog_output: Real | I/Q
      mask Callback t230_QT_dac2_analog_output:
      | validate_analog_data(gcb,230,2,'QT');
      | update_axis_clk(gcb,230);
      mask TypeOptions t230_QT_dac2_inter_mode: 1x | 2x | 4x | 8x | 10x | 12x | 16x | 20x | 24x | 40x
      mask Callback t230_QT_dac2_inter_mode: update_axis_clk(gcb,230);
      mask TypeOptions t230_QT_dac2_sample_per_cycle: 1 | 2 | 3 | 4 | 5 | 6 | 7 | 8 | 9 | 10 | 11 | 12 | 13 | 14 | 15 | 16
      mask Callback t230_QT_dac2_sample_per_cycle: update_axis_clk_label(gcb,230);
      mask TypeOptions t230_QT_dac2_datapath_mode: DUC 0 to Fs/2 | DUC 0 to Fs/4 | DUC Fs/4 to Fs/2 | No DUC 0 to Fs/2
      mask TypeOptions t230_QT_dac2_mixer_type: Bypassed
      mask Callback t230_QT_dac2_mixer_type: mixertype_callback(gcb,230,2,'QT');
      mask TypeOptions t230_QT_dac2_mixer_mode: Real -> Real | I/Q -> Real
      mask Callback t230_QT_dac2_mixer_mode: mixer_callback(gcb,230,2,'QT')
      mask TypeOptions t230_QT_dac2_coarse_freq: 0
      mask TypeOptions t230_QT_dac2_nyquist_zone: Zone 1 | Zone 2
      mask TypeOptions t230_QT_dac2_decode_mode: SNR Optimized | Linearity Optimized
      mask Callback t230_QT_dac3_enable: enable_dac_opt(gcb,230,3);
      mask TypeOptions t230_QT_dac3_analog_output: Real | I/Q
      mask Callback t230_QT_dac3_analog_output:
      | validate_analog_data(gcb,230,3,'QT');
      | update_axis_clk(gcb,230);
      mask TypeOptions t230_QT_dac3_inter_mode: 1x | 2x | 4x | 8x | 10x | 12x | 16x | 20x | 24x | 40x
      mask Callback t230_QT_dac3_inter_mode: update_axis_clk(gcb,230);
      mask TypeOptions t230_QT_dac3_sample_per_cycle: 1 | 2 | 3 | 4 | 5 | 6 | 7 | 8 | 9 | 10 | 11 | 12 | 13 | 14 | 15 | 16
      mask Callback t230_QT_dac3_sample_per_cycle: update_axis_clk_label(gcb,230);
      mask TypeOptions t230_QT_dac3_datapath_mode: DUC 0 to Fs/2 | DUC 0 to Fs/4 | DUC Fs/4 to Fs/2 | No DUC 0 to Fs/2
      mask TypeOptions t230_QT_dac3_mixer_type: Bypassed
      mask Callback t230_QT_dac3_mixer_type: mixertype_callback(gcb,230,3,'QT');
      mask TypeOptions t230_QT_dac3_mixer_mode: Real -> Real | I/Q -> Real
      mask Callback t230_QT_dac3_mixer_mode: mixer_callback(gcb,230,3,'QT')
      mask TypeOptions t230_QT_dac3_coarse_freq: 0
      mask TypeOptions t230_QT_dac3_nyquist_zone: Zone 1 | Zone 2
      mask TypeOptions t230_QT_dac3_decode_mode: SNR Optimized | Linearity Optimized
      mask Callback t231_sample_rate: update_rfdc_clocking(gcb,231);
      mask TypeOptions t231_clk_out: 125 | 62.5 | 31.25 | 15.625
      mask Callback t231_enable_pll:
      | %update_rfdc_clocking(gcb);
      | update_pll(gcb,231);
      mask TypeOptions t231_ref_clk: 923.077 | 857.143 | 800 | 750 | 705.882 | 666.667 | 631.579 | 600 | 571.429 | 545.455 | 521.739 | 500 | 480 | 461.538 | 444.444 | 428.571 | 413.793 | 400 | 387.097 | 375 | 363.636 | 352.941 | 342.857 | 333.333 | 324.324 | 315.789 | 307.692 | 300 | 292.683 | 285.714 | 279.07 | 272.727 | 266.667 | 260.87 | 255.319 | 250 | 244.898 | 240 | 235.294 | 230.769 | 226.415 | 222.222 | 218.182 | 214.286 | 210.526 | 206.897 | 203.39 | 200 | 196.721 | 193.548 | 190.476 | 187.5 | 184.615 | 181.818 | 179.104 | 176.471 | 173.913 | 171.429 | 169.014 | 166.667 | 164.384 | 162.162 | 160 | 157.895 | 155.844 | 153.846 | 151.899 | 150 | 148.148 | 146.341 | 144.578 | 142.857 | 141.176 | 139.535 | 137.931 | 136.364 | 134.831 | 133.333 | 131.868 | 130.435 | 129.032 | 127.66 | 126.316 | 125 | 123.711 | 122.449 | 121.212 | 120 | 118.812 | 117.647 | 116.505 | 115.385 | 114.286 | 113.208 | 112.15 | 111.111 | 110.092 | 109.091 | 108.108 | 107.143 | 106.195 | 105.263 | 104.348 | 103.448 | 102.564
      mask Callback t231_QT_dac0_enable: enable_dac_opt(gcb,231,0);
      mask TypeOptions t231_QT_dac0_analog_output: Real | I/Q
      mask Callback t231_QT_dac0_analog_output:
      | validate_analog_data(gcb,231,0,'QT');
      | update_axis_clk(gcb,231);
      mask TypeOptions t231_QT_dac0_inter_mode: 1x | 2x | 4x | 8x | 10x | 12x | 16x | 20x | 24x | 40x
      mask Callback t231_QT_dac0_inter_mode: update_axis_clk(gcb,231);
      mask TypeOptions t231_QT_dac0_sample_per_cycle: 1 | 2 | 3 | 4 | 5 | 6 | 7 | 8 | 9 | 10 | 11 | 12 | 13 | 14 | 15 | 16
      mask Callback t231_QT_dac0_sample_per_cycle:
      | %update_axis_clk(gcb);
      | update_axis_clk_label(gcb,231);
      mask TypeOptions t231_QT_dac0_datapath_mode: DUC 0 to Fs/2 | DUC 0 to Fs/4 | DUC Fs/4 to Fs/2 | No DUC 0 to Fs/2
      mask TypeOptions t231_QT_dac0_mixer_type: Bypassed
      mask Callback t231_QT_dac0_mixer_type: mixertype_callback(gcb,231,0,'QT');
      mask TypeOptions t231_QT_dac0_mixer_mode: Real -> Real | I/Q -> Real
      mask Callback t231_QT_dac0_mixer_mode: mixer_callback(gcb,231,0,'QT');
      mask TypeOptions t231_QT_dac0_coarse_freq: 0
      mask TypeOptions t231_QT_dac0_nyquist_zone: Zone 1 | Zone 2
      mask TypeOptions t231_QT_dac0_decode_mode: SNR Optimized | Linearity Optimized
      mask Callback t231_QT_dac1_enable: enable_dac_opt(gcb,231,1);
      mask TypeOptions t231_QT_dac1_analog_output: Real | I/Q
      mask Callback t231_QT_dac1_analog_output:
      | validate_analog_data(gcb,231,1,'QT');
      | update_axis_clk(gcb,231);
      mask TypeOptions t231_QT_dac1_inter_mode: 1x | 2x | 4x | 8x | 10x | 12x | 16x | 20x | 24x | 40x
      mask Callback t231_QT_dac1_inter_mode: update_axis_clk(gcb,231);
      mask TypeOptions t231_QT_dac1_sample_per_cycle: 1 | 2 | 3 | 4 | 5 | 6 | 7 | 8 | 9 | 10 | 11 | 12 | 13 | 14 | 15 | 16
      mask Callback t231_QT_dac1_sample_per_cycle: update_axis_clk_label(gcb,231);
      mask TypeOptions t231_QT_dac1_datapath_mode: DUC 0 to Fs/2 | DUC 0 to Fs/4 | DUC Fs/4 to Fs/2 | No DUC 0 to Fs/2
      mask TypeOptions t231_QT_dac1_mixer_type: Bypassed
      mask Callback t231_QT_dac1_mixer_type: mixertype_callback(gcb,231,1,'QT');
      mask TypeOptions t231_QT_dac1_mixer_mode: Real -> Real | I/Q -> Real
      mask Callback t231_QT_dac1_mixer_mode: mixer_callback(gcb,231,1,'QT')
      mask TypeOptions t231_QT_dac1_coarse_freq: 0
      mask TypeOptions t231_QT_dac1_nyquist_zone: Zone 1 | Zone 2
      mask TypeOptions t231_QT_dac1_decode_mode: SNR Optimized | Linearity Optimized
      mask Callback t231_QT_dac2_enable: enable_dac_opt(gcb,231,2);
      mask TypeOptions t231_QT_dac2_analog_output: Real | I/Q
      mask Callback t231_QT_dac2_analog_output:
      | validate_analog_data(gcb,231,2,'QT');
      | update_axis_clk(gcb,231);
      mask TypeOptions t231_QT_dac2_inter_mode: 1x | 2x | 4x | 8x | 10x | 12x | 16x | 20x | 24x | 40x
      mask Callback t231_QT_dac2_inter_mode: update_axis_clk(gcb,231);
      mask TypeOptions t231_QT_dac2_sample_per_cycle: 1 | 2 | 3 | 4 | 5 | 6 | 7 | 8 | 9 | 10 | 11 | 12 | 13 | 14 | 15 | 16
      mask Callback t231_QT_dac2_sample_per_cycle: update_axis_clk_label(gcb,231);
      mask TypeOptions t231_QT_dac2_datapath_mode: DUC 0 to Fs/2 | DUC 0 to Fs/4 | DUC Fs/4 to Fs/2 | No DUC 0 to Fs/2
      mask TypeOptions t231_QT_dac2_mixer_type: Bypassed
      mask Callback t231_QT_dac2_mixer_type: mixertype_callback(gcb,231,2,'QT');
      mask TypeOptions t231_QT_dac2_mixer_mode: Real -> Real | I/Q -> Real
      mask Callback t231_QT_dac2_mixer_mode: mixer_callback(gcb,231,2,'QT')
      mask TypeOptions t231_QT_dac2_coarse_freq: 0
      mask TypeOptions t231_QT_dac2_nyquist_zone: Zone 1 | Zone 2
      mask TypeOptions t231_QT_dac2_decode_mode: SNR Optimized | Linearity Optimized
      mask Callback t231_QT_dac3_enable: enable_dac_opt(gcb,231,3);
      mask TypeOptions t231_QT_dac3_analog_output: Real | I/Q
      mask Callback t231_QT_dac3_analog_output:
      | validate_analog_data(gcb,231,3,'QT');
      | update_axis_clk(gcb,231);
      mask TypeOptions t231_QT_dac3_inter_mode: 1x | 2x | 4x | 8x | 10x | 12x | 16x | 20x | 24x | 40x
      mask Callback t231_QT_dac3_inter_mode: update_axis_clk(gcb,231);
      mask TypeOptions t231_QT_dac3_sample_per_cycle: 1 | 2 | 3 | 4 | 5 | 6 | 7 | 8 | 9 | 10 | 11 | 12 | 13 | 14 | 15 | 16
      mask Callback t231_QT_dac3_sample_per_cycle: update_axis_clk_label(gcb,231);
      mask TypeOptions t231_QT_dac3_datapath_mode: DUC 0 to Fs/2 | DUC 0 to Fs/4 | DUC Fs/4 to Fs/2 | No DUC 0 to Fs/2
      mask TypeOptions t231_QT_dac3_mixer_type: Bypassed
      mask Callback t231_QT_dac3_mixer_type: mixertype_callback(gcb,231,3,'QT');
      mask TypeOptions t231_QT_dac3_mixer_mode: Real -> Real | I/Q -> Real
      mask Callback t231_QT_dac3_mixer_mode: mixer_callback(gcb,231,3,'QT')
      mask TypeOptions t231_QT_dac3_coarse_freq: 0
      mask TypeOptions t231_QT_dac3_nyquist_zone: Zone 1 | Zone 2
      mask TypeOptions t231_QT_dac3_decode_mode: SNR Optimized | Linearity Optimized
      mask TypeOptions t224_adc_clk_src: 224 | 225 | 226 | 227 | 228 | 229 | 230 | 231
      mask TypeOptions t224_clk_dist: None | Input Refclk | PLL Output
      mask TypeOptions t225_adc_clk_src: 224 | 225 | 226 | 227 | 228 | 229 | 230 | 231
      mask TypeOptions t225_clk_dist: None | Input Refclk | PLL Output
      mask TypeOptions t226_adc_clk_src: 224 | 225 | 226 | 227 | 228 | 229 | 230 | 231
      mask TypeOptions t226_clk_dist: None | Input Refclk | PLL Output
      mask TypeOptions t227_adc_clk_src: 224 | 225 | 226 | 227 | 228 | 229 | 230 | 231
      mask TypeOptions t227_clk_dist: None | Input Refclk | PLL Output
      mask TypeOptions t228_dac_clk_src: 224 | 225 | 226 | 227 | 228 | 229 | 230 | 231
      mask TypeOptions t228_clk_dist: None | Input Refclk | PLL Output
      mask TypeOptions t229_dac_clk_src: 224 | 225 | 226 | 227 | 228 | 229 | 230 | 231
      mask TypeOptions t229_clk_dist: None | Input Refclk | PLL Output
      mask TypeOptions t230_dac_clk_src: 224 | 225 | 226 | 227 | 228 | 229 | 230 | 231
      mask TypeOptions t230_clk_dist: None | Input Refclk | PLL Output
      mask TypeOptions t231_dac_clk_src: 224 | 225 | 226 | 227 | 228 | 229 | 230 | 231
      mask TypeOptions t231_clk_dist: None | Input Refclk | PLL Output
      mask Callback maskdoneopening:
      | %assignin('base','mask_opening',0)
      | %assignin('base','run_init',1)
      | set_param(gcb,'maskopening','0')
      | set_param(gcb,'runinit','1')
      mask DialogControl ADCTileSelect Prompt: ADC Tiles
      mask DialogControl Tile224_container Prompt: Tile 224
      mask DialogControl pll_clocking_config_224 Prompt: Clocking and PLL Configuration
      mask DialogControl t224_QuadTileConfig Prompt: Quad Tile Configuration
      mask DialogControl t224_ADCPair01 Prompt: ADC Pair 0,1
      mask DialogControl t224_QT_adc0 Prompt: ADC 0
      mask DialogControl t224_QT_adc0_DataSettings Prompt: Data Settings
      mask DialogControl t224_QT_adc0_req_axis_clk_label Prompt: Required AXI4-Stream clock:
      mask DialogControl t224_QT_adc0_MixerSettings Prompt: MIxer Settings
      mask DialogControl t224_QT_adc0_AnalogSettings Prompt: Analog Settings
      mask DialogControl t224_QT_adc1 Prompt: ADC 1
      mask DialogControl t224_QT_adc1_DataSettings Prompt: Data Settings
      mask DialogControl t224_QT_adc1_req_axis_clk_label Prompt: Required AXI4-Stream clock:
      mask DialogControl t224_QT_adc1_MixerSettings Prompt: MIxer Settings
      mask DialogControl t224_QT_adc1_AnalogSettings Prompt: Analog Settings
      mask DialogControl ADCPair23 Prompt: ADC Pair 2,3
      mask DialogControl QT_adc2 Prompt: ADC 2
      mask DialogControl t224_QT_adc2_DataSettings Prompt: Data Settings
      mask DialogControl t224_QT_adc2_req_axis_clk_label Prompt: Required AXI4-Stream clock:
      mask DialogControl t224_QT_adc2_MixerSettings Prompt: MIxer Settings
      mask DialogControl t224_QT_adc2_AnalogSettings Prompt: Analog Settings
      mask DialogControl t224_QT_adc3 Prompt: ADC 3
      mask DialogControl t224_QT_adc3_DataSettings Prompt: Data Settings
      mask DialogControl t224_QT_adc3_req_axis_clk_label Prompt: Required AXI4-Stream clock:
      mask DialogControl t224_QT_adc3_MixerSettings Prompt: MIxer Settings
      mask DialogControl t224_QT_adc3_AnalogSettings Prompt: Analog Settings
      mask DialogControl t224_DualTileConfig Prompt: Dual Tile Configuration
      mask DialogControl t224_DT_adc0 Prompt: ADC 0
      mask DialogControl t224_DT_adc0_DataSettings Prompt: Data Settings
      mask DialogControl t224_DT_adc0_req_axis_clk_label Prompt: Required AXI4-Stream clock:
      mask DialogControl t224_DT_adc0_MixerSettings Prompt: MIxer Settings
      mask DialogControl t224_DT_adc0_AnalogSettings Prompt: Analog Settings
      mask DialogControl t224_DT_adc1 Prompt: ADC 1
      mask DialogControl t224_DT_adc1_DataSettings Prompt: Data Settings
      mask DialogControl t224_DT_adc1_req_axis_clk_label Prompt: Required AXI4-Stream clock:
      mask DialogControl t224_DT_adc1_MixerSettings Prompt: MIxer Settings
      mask DialogControl t224_DT_adc1_AnalogSettings Prompt: Analog Settings
      mask DialogControl Tile225_container Prompt: Tile 225
      mask DialogControl pll_clocking_config_225 Prompt: Clocking and PLL Configuration
      mask DialogControl t225_QuadTileConfig Prompt: Quad Tile Configuration
      mask DialogControl t225_ADCPair01 Prompt: ADC Pair 0,1
      mask DialogControl t225_QT_adc0 Prompt: ADC 0
      mask DialogControl t225_QT_adc0_DataSettings Prompt: Data Settings
      mask DialogControl t225_QT_adc0_req_axis_clk_label Prompt: Required AXI4-Stream clock:
      mask DialogControl t225_QT_adc0_MixerSettings Prompt: MIxer Settings
      mask DialogControl t225_QT_adc0_AnalogSettings Prompt: Analog Settings
      mask DialogControl t225_QT_adc1 Prompt: ADC 1
      mask DialogControl t225_QT_adc1_DataSettings Prompt: Data Settings
      mask DialogControl t225_QT_adc1_req_axis_clk_label Prompt: Required AXI4-Stream clock:
      mask DialogControl t225_QT_adc1_MixerSettings Prompt: MIxer Settings
      mask DialogControl t225_QT_adc1_AnalogSettings Prompt: Analog Settings
      mask DialogControl t225_ADCPair23 Prompt: ADC Pair 2,3
      mask DialogControl t225_QT_adc2 Prompt: ADC 2
      mask DialogControl t225_QT_adc2_DataSettings Prompt: Data Settings
      mask DialogControl t225_QT_adc2_req_axis_clk_label Prompt: Required AXI4-Stream clock:
      mask DialogControl t225_QT_adc2_MixerSettings Prompt: MIxer Settings
      mask DialogControl t225_QT_adc2_AnalogSettings Prompt: Analog Settings
      mask DialogControl t225_QT_adc3 Prompt: ADC 3
      mask DialogControl t225_QT_adc3_DataSettings Prompt: Data Settings
      mask DialogControl t225_QT_adc3_req_axis_clk_label Prompt: Required AXI4-Stream clock:
      mask DialogControl t225_QT_adc3_MixerSettings Prompt: MIxer Settings
      mask DialogControl t225_QT_adc3_AnalogSettings Prompt: Analog Settings
      mask DialogControl t225_DualTileConfig Prompt: Dual Tile Configuration
      mask DialogControl t225_DT_adc0 Prompt: ADC 0
      mask DialogControl t225_DT_adc0_DataSettings Prompt: Data Settings
      mask DialogControl t225_DT_adc0_req_axis_clk_label Prompt: Required AXI4-Stream clock:
      mask DialogControl t225_DT_adc0_MixerSettings Prompt: MIxer Settings
      mask DialogControl t225_DT_adc0_AnalogSettings Prompt: Analog Settings
      mask DialogControl t225_DT_adc1 Prompt: ADC 1
      mask DialogControl t225_DT_adc1_DataSettings Prompt: Data Settings
      mask DialogControl t225_DT_adc1_req_axis_clk_label Prompt: Required AXI4-Stream clock:
      mask DialogControl t225_DT_adc1_MixerSettings Prompt: MIxer Settings
      mask DialogControl t225_DT_adc1_AnalogSettings Prompt: Analog Settings
      mask DialogControl Tile226_container Prompt: Tile 226
      mask DialogControl pll_clocking_config_226 Prompt: Clocking and PLL Configuration
      mask DialogControl t226_QuadTileConfig Prompt: Quad Tile Configuration
      mask DialogControl t226_ADCPair01 Prompt: ADC Pair 0,1
      mask DialogControl t226_QT_adc0 Prompt: ADC 0
      mask DialogControl t226_QT_adc0_DataSettings Prompt: Data Settings
      mask DialogControl t226_QT_adc0_req_axis_clk_label Prompt: Required AXI4-Stream clock:
      mask DialogControl t226_QT_adc0_MixerSettings Prompt: MIxer Settings
      mask DialogControl t226_QT_adc0_AnalogSettings Prompt: Analog Settings
      mask DialogControl t226_QT_adc1 Prompt: ADC 1
      mask DialogControl t226_QT_adc1_DataSettings Prompt: Data Settings
      mask DialogControl t226_QT_adc1_req_axis_clk_label Prompt: Required AXI4-Stream clock:
      mask DialogControl t226_QT_adc1_MixerSettings Prompt: MIxer Settings
      mask DialogControl t226_QT_adc1_AnalogSettings Prompt: Analog Settings
      mask DialogControl t226_ADCPair23 Prompt: ADC Pair 2,3
      mask DialogControl t226_QT_adc2 Prompt: ADC 2
      mask DialogControl t226_QT_adc2_DataSettings Prompt: Data Settings
      mask DialogControl t226_QT_adc2_req_axis_clk_label Prompt: Required AXI4-Stream clock:
      mask DialogControl t226_QT_adc2_MixerSettings Prompt: MIxer Settings
      mask DialogControl t226_QT_adc2_AnalogSettings Prompt: Analog Settings
      mask DialogControl t226_QT_adc3 Prompt: ADC 3
      mask DialogControl t226_QT_adc3_DataSettings Prompt: Data Settings
      mask DialogControl t226_QT_adc3_req_axis_clk_label Prompt: Required AXI4-Stream clock:
      mask DialogControl t226_QT_adc3_MixerSettings Prompt: MIxer Settings
      mask DialogControl t226_QT_adc3_AnalogSettings Prompt: Analog Settings
      mask DialogControl t226_DualTileConfig Prompt: Dual Tile Configuration
      mask DialogControl t226_DT_adc0 Prompt: ADC 0
      mask DialogControl t226_DT_adc0_DataSettings Prompt: Data Settings
      mask DialogControl t226_DT_adc0_req_axis_clk_label Prompt: Required AXI4-Stream clock:
      mask DialogControl t226_DT_adc0_MixerSettings Prompt: MIxer Settings
      mask DialogControl t226_DT_adc0_AnalogSettings Prompt: Analog Settings
      mask DialogControl t226_DT_adc1 Prompt: ADC 1
      mask DialogControl t226_DT_adc1_DataSettings Prompt: Data Settings
      mask DialogControl t226_DT_adc1_req_axis_clk_label Prompt: Required AXI4-Stream clock:
      mask DialogControl t226_DT_adc1_MixerSettings Prompt: MIxer Settings
      mask DialogControl t226_DT_adc1_AnalogSettings Prompt: Analog Settings
      mask DialogControl Tile227_container Prompt: Tile 227
      mask DialogControl pll_clocking_config_227 Prompt: Clocking and PLL Configuration
      mask DialogControl t227_QuadTileConfig Prompt: Quad Tile Configuration
      mask DialogControl t227_ADCPair01 Prompt: ADC Pair 0,1
      mask DialogControl t227_QT_adc0 Prompt: ADC 0
      mask DialogControl t227_QT_adc0_DataSettings Prompt: Data Settings
      mask DialogControl t227_QT_adc0_req_axis_clk_label Prompt: Required AXI4-Stream clock:
      mask DialogControl t227_QT_adc0_MixerSettings Prompt: MIxer Settings
      mask DialogControl t227_QT_adc0_AnalogSettings Prompt: Analog Settings
      mask DialogControl t227_QT_adc1 Prompt: ADC 1
      mask DialogControl t227_QT_adc1_DataSettings Prompt: Data Settings
      mask DialogControl t227_QT_adc1_req_axis_clk_label Prompt: Required AXI4-Stream clock:
      mask DialogControl t227_QT_adc1_MixerSettings Prompt: MIxer Settings
      mask DialogControl t227_QT_adc1_AnalogSettings Prompt: Analog Settings
      mask DialogControl t227_ADCPair23 Prompt: ADC Pair 2,3
      mask DialogControl t227_QT_adc2 Prompt: ADC 2
      mask DialogControl t227_QT_adc2_DataSettings Prompt: Data Settings
      mask DialogControl t227_QT_adc2_req_axis_clk_label Prompt: Required AXI4-Stream clock:
      mask DialogControl t227_QT_adc2_MixerSettings Prompt: MIxer Settings
      mask DialogControl t227_QT_adc2_AnalogSettings Prompt: Analog Settings
      mask DialogControl t227_QT_adc3 Prompt: ADC 3
      mask DialogControl t227_QT_adc3_DataSettings Prompt: Data Settings
      mask DialogControl t227_QT_adc3_req_axis_clk_label Prompt: Required AXI4-Stream clock:
      mask DialogControl t227_QT_adc3_MixerSettings Prompt: MIxer Settings
      mask DialogControl t227_QT_adc3_AnalogSettings Prompt: Analog Settings
      mask DialogControl t227_DualTileConfig Prompt: Dual Tile Configuration
      mask DialogControl t227_DT_adc0 Prompt: ADC 0
      mask DialogControl t227_DT_adc0_DataSettings Prompt: Data Settings
      mask DialogControl t227_DT_adc0_req_axis_clk_label Prompt: Required AXI4-Stream clock:
      mask DialogControl t227_DT_adc0_MixerSettings Prompt: MIxer Settings
      mask DialogControl t227_DT_adc0_AnalogSettings Prompt: Analog Settings
      mask DialogControl t227_DT_adc1 Prompt: ADC 1
      mask DialogControl t227_DT_adc1_DataSettings Prompt: Data Settings
      mask DialogControl t227_DT_adc1_req_axis_clk_label Prompt: Required AXI4-Stream clock:
      mask DialogControl t227_DT_adc1_MixerSettings Prompt: MIxer Settings
      mask DialogControl t227_DT_adc1_AnalogSettings Prompt: Analog Settings
      mask DialogControl DACTileSelect Prompt: DAC Tiles
      mask DialogControl Tile228_container Prompt: Tile 228
      mask DialogControl pll_clocking_config_228 Prompt: Clocking and PLL Configuration
      mask DialogControl t228_QuadTileConfig Prompt: Quad Tile Configuration
      mask DialogControl t228_DACPair01 Prompt: DAC Pair 0,1
      mask DialogControl t228_QT_dac0 Prompt: DAC 0
      mask DialogControl t228_QT_dac0_DataSettings Prompt: Data Settings
      mask DialogControl t228_QT_dac0_req_axis_clk_label Prompt: Required AXI4-Stream clock:
      mask DialogControl t228_QT_dac0_MixerSettings Prompt: MIxer Settings
      mask DialogControl t228_QT_dac0_AnalogSettings Prompt: Analog Settings
      mask DialogControl t228_QT_dac1 Prompt: DAC 1
      mask DialogControl t228_QT_dac1_DataSettings Prompt: Data Settings
      mask DialogControl t228_QT_dac1_req_axis_clk_label Prompt: Required AXI4-Stream clock:
      mask DialogControl t228_QT_dac1_MixerSettings Prompt: MIxer Settings
      mask DialogControl t228_QT_dac1_AnalogSettings Prompt: Analog Settings
      mask DialogControl t228_DACPair23 Prompt: DAC Pair 2,3
      mask DialogControl t228_QT_dac2 Prompt: DAC 2
      mask DialogControl t228_QT_dac2_DataSettings Prompt: Data Settings
      mask DialogControl t228_QT_dac2_req_axis_clk_label Prompt: Required AXI4-Stream clock:
      mask DialogControl t228_QT_dac2_MixerSettings Prompt: MIxer Settings
      mask DialogControl t228_QT_dac2_AnalogSettings Prompt: Analog Settings
      mask DialogControl t228_QT_dac3 Prompt: DAC 3
      mask DialogControl t228_QT_dac3_DataSettings Prompt: Data Settings
      mask DialogControl t228_QT_dac3_req_axis_clk_label Prompt: Required AXI4-Stream clock:
      mask DialogControl t228_QT_dac3_MixerSettings Prompt: MIxer Settings
      mask DialogControl t228_QT_dac3_AnalogSettings Prompt: Analog Settings
      mask DialogControl t228_DualTileConfig Prompt: Dual Tile Configuration
      mask DialogControl t228_DACPair01_DT Prompt: DAC Pair 0,1
      mask DialogControl t228_DT_dac0 Prompt: DAC 0
      mask DialogControl t228_DT_dac0_DataSettings Prompt: Data Settings
      mask DialogControl t228_DT_dac0_req_axis_clk_label Prompt: Required AXI4-Stream clock:
      mask DialogControl t228_DT_dac0_MixerSettings Prompt: MIxer Settings
      mask DialogControl t228_DT_dac0_AnalogSettings Prompt: Analog Settings
      mask DialogControl t228_DT_dac1 Prompt: DAC 1
      mask DialogControl t228_DT_dac1_DataSettings Prompt: Data Settings
      mask DialogControl t228_DT_dac1_req_axis_clk_label Prompt: Required AXI4-Stream clock:
      mask DialogControl t228_DT_dac1_MixerSettings Prompt: MIxer Settings
      mask DialogControl t228_DT_dac1_AnalogSettings Prompt: Analog Settings
      mask DialogControl t228_DACPair23_DT Prompt: DAC Pair 2,3
      mask DialogControl t228_DT_dac2 Prompt: DAC 2
      mask DialogControl t228_DT_dac2_DataSettings Prompt: Data Settings
      mask DialogControl t228_DT_dac2_req_axis_clk_label Prompt: Required AXI4-Stream clock:
      mask DialogControl t228_DT_dac2_MixerSettings Prompt: MIxer Settings
      mask DialogControl t228_DT_dac2_AnalogSettings Prompt: Analog Settings
      mask DialogControl t228_DT_dac3 Prompt: DAC 3
      mask DialogControl t228_DT_dac3_DataSettings Prompt: Data Settings
      mask DialogControl t228_DT_dac3_req_axis_clk_label Prompt: Required AXI4-Stream clock:
      mask DialogControl t228_DT_dac3_MixerSettings Prompt: MIxer Settings
      mask DialogControl t228_DT_dac3_AnalogSettings Prompt: Analog Settings
      mask DialogControl Tile229_container Prompt: Tile 229
      mask DialogControl pll_clocking_config_229 Prompt: Clocking and PLL Configuration
      mask DialogControl t229_QuadTileConfig Prompt: Quad Tile Configuration
      mask DialogControl t229_DACPair01 Prompt: DAC Pair 0,1
      mask DialogControl t229_QT_dac0 Prompt: DAC 0
      mask DialogControl t229_QT_dac0_DataSettings Prompt: Data Settings
      mask DialogControl t229_QT_dac0_req_axis_clk_label Prompt: Required AXI4-Stream clock:
      mask DialogControl t229_QT_dac0_MixerSettings Prompt: MIxer Settings
      mask DialogControl t229_QT_dac0_AnalogSettings Prompt: Analog Settings
      mask DialogControl t229_QT_dac1 Prompt: DAC 1
      mask DialogControl t229_QT_dac1_DataSettings Prompt: Data Settings
      mask DialogControl t229_QT_dac1_req_axis_clk_label Prompt: Required AXI4-Stream clock:
      mask DialogControl t229_QT_dac1_MixerSettings Prompt: MIxer Settings
      mask DialogControl t229_QT_dac1_AnalogSettings Prompt: Analog Settings
      mask DialogControl t229_DACPair23 Prompt: DAC Pair 2,3
      mask DialogControl t229_QT_dac2 Prompt: DAC 2
      mask DialogControl t229_QT_dac2_DataSettings Prompt: Data Settings
      mask DialogControl t229_QT_dac2_req_axis_clk_label Prompt: Required AXI4-Stream clock:
      mask DialogControl t229_QT_dac2_MixerSettings Prompt: MIxer Settings
      mask DialogControl t229_QT_dac2_AnalogSettings Prompt: Analog Settings
      mask DialogControl t229_QT_dac3 Prompt: DAC 3
      mask DialogControl t229_QT_dac3_DataSettings Prompt: Data Settings
      mask DialogControl t229_QT_dac3_req_axis_clk_label Prompt: Required AXI4-Stream clock:
      mask DialogControl t229_QT_dac3_MixerSettings Prompt: MIxer Settings
      mask DialogControl t229_QT_dac3_AnalogSettings Prompt: Analog Settings
      mask DialogControl t229_DualTileConfig Prompt: Dual Tile Configuration
      mask DialogControl t229_DACPair01_DT Prompt: DAC Pair 0,1
      mask DialogControl t229_DT_dac0 Prompt: DAC 0
      mask DialogControl t229_DT_dac0_DataSettings Prompt: Data Settings
      mask DialogControl t229_DT_dac0_req_axis_clk_label Prompt: Required AXI4-Stream clock:
      mask DialogControl t229_DT_dac0_MixerSettings Prompt: MIxer Settings
      mask DialogControl t229_DT_dac0_AnalogSettings Prompt: Analog Settings
      mask DialogControl t229_DT_dac1 Prompt: DAC 1
      mask DialogControl t229_DT_dac1_DataSettings Prompt: Data Settings
      mask DialogControl t229_DT_dac1_req_axis_clk_label Prompt: Required AXI4-Stream clock:
      mask DialogControl t229_DT_dac1_MixerSettings Prompt: MIxer Settings
      mask DialogControl t229_DT_dac1_AnalogSettings Prompt: Analog Settings
      mask DialogControl t229_DACPair23_DT Prompt: DAC Pair 2,3
      mask DialogControl t229_DT_dac2 Prompt: DAC 2
      mask DialogControl t229_DT_dac2_DataSettings Prompt: Data Settings
      mask DialogControl t229_DT_dac2_req_axis_clk_label Prompt: Required AXI4-Stream clock:
      mask DialogControl t229_DT_dac2_MixerSettings Prompt: MIxer Settings
      mask DialogControl t229_DT_dac2_AnalogSettings Prompt: Analog Settings
      mask DialogControl t229_DT_dac3 Prompt: DAC 3
      mask DialogControl t229_DT_dac3_DataSettings Prompt: Data Settings
      mask DialogControl t229_DT_dac3_req_axis_clk_label Prompt: Required AXI4-Stream clock:
      mask DialogControl t229_DT_dac3_MixerSettings Prompt: MIxer Settings
      mask DialogControl t229_DT_dac3_AnalogSettings Prompt: Analog Settings
      mask DialogControl Tile230_container Prompt: Tile 230
      mask DialogControl pll_clocking_config_230 Prompt: Clocking and PLL Configuration
      mask DialogControl t230_QuadTileConfig Prompt: Quad Tile Configuration
      mask DialogControl t230_DACPair01 Prompt: DAC Pair 0,1
      mask DialogControl t230_QT_dac0 Prompt: DAC 0
      mask DialogControl t230_QT_dac0_DataSettings Prompt: Data Settings
      mask DialogControl t230_QT_dac0_req_axis_clk_label Prompt: Required AXI4-Stream clock:
      mask DialogControl t230_QT_dac0_MixerSettings Prompt: MIxer Settings
      mask DialogControl t230_QT_dac0_AnalogSettings Prompt: Analog Settings
      mask DialogControl t230_QT_dac1 Prompt: DAC 1
      mask DialogControl t230_QT_dac1_DataSettings Prompt: Data Settings
      mask DialogControl t230_QT_dac1_req_axis_clk_label Prompt: Required AXI4-Stream clock:
      mask DialogControl t230_QT_dac1_MixerSettings Prompt: MIxer Settings
      mask DialogControl t230_QT_dac1_AnalogSettings Prompt: Analog Settings
      mask DialogControl t230_DACPair23 Prompt: DAC Pair 2,3
      mask DialogControl t230_QT_dac2 Prompt: DAC 2
      mask DialogControl t230_QT_dac2_DataSettings Prompt: Data Settings
      mask DialogControl t230_QT_dac2_req_axis_clk_label Prompt: Required AXI4-Stream clock:
      mask DialogControl t230_QT_dac2_MixerSettings Prompt: MIxer Settings
      mask DialogControl t230_QT_dac2_AnalogSettings Prompt: Analog Settings
      mask DialogControl t230_QT_dac3 Prompt: DAC 3
      mask DialogControl t230_QT_dac3_DataSettings Prompt: Data Settings
      mask DialogControl t230_QT_dac3_req_axis_clk_label Prompt: Required AXI4-Stream clock:
      mask DialogControl t230_QT_dac3_MixerSettings Prompt: MIxer Settings
      mask DialogControl t230_QT_dac3_AnalogSettings Prompt: Analog Settings
      mask DialogControl t230_DualTileConfig Prompt: Dual Tile Configuration
      mask DialogControl Control58 Prompt: Tile 230 does not exist for DT configs
      mask DialogControl Tile231_container Prompt: Tile 231
      mask DialogControl pll_clocking_config_231 Prompt: Clocking and PLL Configuration
      mask DialogControl t231_QuadTileConfig Prompt: Quad Tile Configuration
      mask DialogControl t231_DACPair01 Prompt: DAC Pair 0,1
      mask DialogControl t231_QT_dac0 Prompt: DAC 0
      mask DialogControl t231_QT_dac0_DataSettings Prompt: Data Settings
      mask DialogControl t231_QT_dac0_req_axis_clk_label Prompt: Required AXI4-Stream clock:
      mask DialogControl t231_QT_dac0_MixerSettings Prompt: MIxer Settings
      mask DialogControl t231_QT_dac0_AnalogSettings Prompt: Analog Settings
      mask DialogControl t231_QT_dac1 Prompt: DAC 1
      mask DialogControl t231_QT_dac1_DataSettings Prompt: Data Settings
      mask DialogControl t231_QT_dac1_req_axis_clk_label Prompt: Required AXI4-Stream clock:
      mask DialogControl t231_QT_dac1_MixerSettings Prompt: MIxer Settings
      mask DialogControl t231_QT_dac1_AnalogSettings Prompt: Analog Settings
      mask DialogControl t231_DACPair23 Prompt: DAC Pair 2,3
      mask DialogControl t231_QT_dac2 Prompt: DAC 2
      mask DialogControl t231_QT_dac2_DataSettings Prompt: Data Settings
      mask DialogControl t231_QT_dac2_req_axis_clk_label Prompt: Required AXI4-Stream clock:
      mask DialogControl t231_QT_dac2_MixerSettings Prompt: MIxer Settings
      mask DialogControl t231_QT_dac2_AnalogSettings Prompt: Analog Settings
      mask DialogControl t231_QT_dac3 Prompt: DAC 3
      mask DialogControl t231_QT_dac3_DataSettings Prompt: Data Settings
      mask DialogControl t231_QT_dac3_req_axis_clk_label Prompt: Required AXI4-Stream clock:
      mask DialogControl t231_QT_dac3_MixerSettings Prompt: MIxer Settings
      mask DialogControl t231_QT_dac3_AnalogSettings Prompt: Analog Settings
      mask DialogControl t231_DualTileConfig Prompt: Dual Tile Configuration
      mask DialogControl Control59 Prompt: Tile 231 does not exist for DT configs
      mask DialogControl SystemClocking Prompt: System Clocking
      mask DialogControl ADCClocking Prompt: ADC Tile Clocking
      mask DialogControl t224_clock_config Prompt: ADC Tile 0
      mask DialogControl t225_clock_config Prompt: ADC Tile 1
      mask DialogControl t226_clock_config Prompt: ADC Tile 2
      mask DialogControl t227_clock_config Prompt: ADC Tile 3
      mask DialogControl DACClocking Prompt: DAC Tile Clocking
      mask DialogControl t228_clock_config Prompt: DAC Tile 0
      mask DialogControl t229_clock_config Prompt: DAC Tile 1
      mask DialogControl t230_clock_config Prompt: DAC Tile 2
      mask DialogControl t231_clock_config Prompt: DAC Tile 3
